simulink model "H175_V2_control"  (R2025b)
(part 2 of 12)

  ct_R_index3 : nesl_utility/Simulink-PS Converter  PhysicalDomain=network_engine_domain  SubClassName=ps_input  LeftPortType=input  RightPortType=output  PseudoPeriodic=off  Frequencies=[]  NoiseDistribution=none  NoiseParameters=[]  Unit=N*m  AffineConversion=off  FilteringAndDerivatives=provide  SimscapeFilterOrder=1  InputFilterTimeConstant=0.001  UdotUserProvided=0
  ct_R_little1 : nesl_utility/Simulink-PS Converter  PhysicalDomain=network_engine_domain  SubClassName=ps_input  LeftPortType=input  RightPortType=output  PseudoPeriodic=off  Frequencies=[]  NoiseDistribution=none  NoiseParameters=[]  Unit=N*m  AffineConversion=off  FilteringAndDerivatives=provide  SimscapeFilterOrder=1  InputFilterTimeConstant=0.001  UdotUserProvided=0
  ct_R_little2 : nesl_utility/Simulink-PS Converter  PhysicalDomain=network_engine_domain  SubClassName=ps_input  LeftPortType=input  RightPortType=output  PseudoPeriodic=off  Frequencies=[]  NoiseDistribution=none  NoiseParameters=[]  Unit=N*m  AffineConversion=off  FilteringAndDerivatives=provide  SimscapeFilterOrder=1  InputFilterTimeConstant=0.001  UdotUserProvided=0
  ct_R_little3 : nesl_utility/Simulink-PS Converter  PhysicalDomain=network_engine_domain  SubClassName=ps_input  LeftPortType=input  RightPortType=output  PseudoPeriodic=off  Frequencies=[]  NoiseDistribution=none  NoiseParameters=[]  Unit=N*m  AffineConversion=off  FilteringAndDerivatives=provide  SimscapeFilterOrder=1  InputFilterTimeConstant=0.001  UdotUserProvided=0
  ct_R_middle1 : nesl_utility/Simulink-PS Converter  PhysicalDomain=network_engine_domain  SubClassName=ps_input  LeftPortType=input  RightPortType=output  PseudoPeriodic=off  Frequencies=[]  NoiseDistribution=none  NoiseParameters=[]  Unit=N*m  AffineConversion=off  FilteringAndDerivatives=provide  SimscapeFilterOrder=1  InputFilterTimeConstant=0.001  UdotUserProvided=0
  ct_R_middle2 : nesl_utility/Simulink-PS Converter  PhysicalDomain=network_engine_domain  SubClassName=ps_input  LeftPortType=input  RightPortType=output  PseudoPeriodic=off  Frequencies=[]  NoiseDistribution=none  NoiseParameters=[]  Unit=N*m  AffineConversion=off  FilteringAndDerivatives=provide  SimscapeFilterOrder=1  InputFilterTimeConstant=0.001  UdotUserProvided=0
  ct_R_middle3 : nesl_utility/Simulink-PS Converter  PhysicalDomain=network_engine_domain  SubClassName=ps_input  LeftPortType=input  RightPortType=output  PseudoPeriodic=off  Frequencies=[]  NoiseDistribution=none  NoiseParameters=[]  Unit=N*m  AffineConversion=off  FilteringAndDerivatives=provide  SimscapeFilterOrder=1  InputFilterTimeConstant=0.001  UdotUserProvided=0
  ct_R_ring1 : nesl_utility/Simulink-PS Converter  PhysicalDomain=network_engine_domain  SubClassName=ps_input  LeftPortType=input  RightPortType=output  PseudoPeriodic=off  Frequencies=[]  NoiseDistribution=none  NoiseParameters=[]  Unit=N*m  AffineConversion=off  FilteringAndDerivatives=provide  SimscapeFilterOrder=1  InputFilterTimeConstant=0.001  UdotUserProvided=0
  ct_R_ring2 : nesl_utility/Simulink-PS Converter  PhysicalDomain=network_engine_domain  SubClassName=ps_input  LeftPortType=input  RightPortType=output  PseudoPeriodic=off  Frequencies=[]  NoiseDistribution=none  NoiseParameters=[]  Unit=N*m  AffineConversion=off  FilteringAndDerivatives=provide  SimscapeFilterOrder=1  InputFilterTimeConstant=0.001  UdotUserProvided=0
  ct_R_ring3 : nesl_utility/Simulink-PS Converter  PhysicalDomain=network_engine_domain  SubClassName=ps_input  LeftPortType=input  RightPortType=output  PseudoPeriodic=off  Frequencies=[]  NoiseDistribution=none  NoiseParameters=[]  Unit=N*m  AffineConversion=off  FilteringAndDerivatives=provide  SimscapeFilterOrder=1  InputFilterTimeConstant=0.001  UdotUserProvided=0
  ct_R_scapula : nesl_utility/Simulink-PS Converter  PhysicalDomain=network_engine_domain  SubClassName=ps_input  LeftPortType=input  RightPortType=output  PseudoPeriodic=off  Frequencies=[]  NoiseDistribution=none  NoiseParameters=[]  Unit=N*m  AffineConversion=off  FilteringAndDerivatives=provide  SimscapeFilterOrder=1  InputFilterTimeConstant=0.001  UdotUserProvided=0
  ct_R_shin : nesl_utility/Simulink-PS Converter  PhysicalDomain=network_engine_domain  SubClassName=ps_input  LeftPortType=input  RightPortType=output  PseudoPeriodic=off  Frequencies=[]  NoiseDistribution=none  NoiseParameters=[]  Unit=N*m  AffineConversion=off  FilteringAndDerivatives=provide  SimscapeFilterOrder=1  InputFilterTimeConstant=0.001  UdotUserProvided=0
  ct_R_shoulder_roll : nesl_utility/Simulink-PS Converter  PhysicalDomain=network_engine_domain  SubClassName=ps_input  LeftPortType=input  RightPortType=output  PseudoPeriodic=off  Frequencies=[]  NoiseDistribution=none  NoiseParameters=[]  Unit=N*m  AffineConversion=off  FilteringAndDerivatives=provide  SimscapeFilterOrder=1  InputFilterTimeConstant=0.001  UdotUserProvided=0
  ct_R_shoulder_yaw : nesl_utility/Simulink-PS Converter  PhysicalDomain=network_engine_domain  SubClassName=ps_input  LeftPortType=input  RightPortType=output  PseudoPeriodic=off  Frequencies=[]  NoiseDistribution=none  NoiseParameters=[]  Unit=N*m  AffineConversion=off  FilteringAndDerivatives=provide  SimscapeFilterOrder=1  InputFilterTimeConstant=0.001  UdotUserProvided=0
  ct_R_thigh : nesl_utility/Simulink-PS Converter  PhysicalDomain=network_engine_domain  SubClassName=ps_input  LeftPortType=input  RightPortType=output  PseudoPeriodic=off  Frequencies=[]  NoiseDistribution=none  NoiseParameters=[]  Unit=N*m  AffineConversion=off  FilteringAndDerivatives=provide  SimscapeFilterOrder=1  InputFilterTimeConstant=0.001  UdotUserProvided=0
  ct_R_thumb1 : nesl_utility/Simulink-PS Converter  PhysicalDomain=network_engine_domain  SubClassName=ps_input  LeftPortType=input  RightPortType=output  PseudoPeriodic=off  Frequencies=[]  NoiseDistribution=none  NoiseParameters=[]  Unit=N*m  AffineConversion=off  FilteringAndDerivatives=provide  SimscapeFilterOrder=1  InputFilterTimeConstant=0.001  UdotUserProvided=0
  ct_R_thumb2 : nesl_utility/Simulink-PS Converter  PhysicalDomain=network_engine_domain  SubClassName=ps_input  LeftPortType=input  RightPortType=output  PseudoPeriodic=off  Frequencies=[]  NoiseDistribution=none  NoiseParameters=[]  Unit=N*m  AffineConversion=off  FilteringAndDerivatives=provide  SimscapeFilterOrder=1  InputFilterTimeConstant=0.001  UdotUserProvided=0
  ct_R_thumb3 : nesl_utility/Simulink-PS Converter  PhysicalDomain=network_engine_domain  SubClassName=ps_input  LeftPortType=input  RightPortType=output  PseudoPeriodic=off  Frequencies=[]  NoiseDistribution=none  NoiseParameters=[]  Unit=N*m  AffineConversion=off  FilteringAndDerivatives=provide  SimscapeFilterOrder=1  InputFilterTimeConstant=0.001  UdotUserProvided=0
  ct_R_toe : nesl_utility/Simulink-PS Converter  PhysicalDomain=network_engine_domain  SubClassName=ps_input  LeftPortType=input  RightPortType=output  PseudoPeriodic=off  Frequencies=[]  NoiseDistribution=none  NoiseParameters=[]  Unit=N*m  AffineConversion=off  FilteringAndDerivatives=provide  SimscapeFilterOrder=1  InputFilterTimeConstant=0.001  UdotUserProvided=0
  ct_R_upper_arm : nesl_utility/Simulink-PS Converter  PhysicalDomain=network_engine_domain  SubClassName=ps_input  LeftPortType=input  RightPortType=output  PseudoPeriodic=off  Frequencies=[]  NoiseDistribution=none  NoiseParameters=[]  Unit=N*m  AffineConversion=off  FilteringAndDerivatives=provide  SimscapeFilterOrder=1  InputFilterTimeConstant=0.001  UdotUserProvided=0
  ct_R_wrist_roll : nesl_utility/Simulink-PS Converter  PhysicalDomain=network_engine_domain  SubClassName=ps_input  LeftPortType=input  RightPortType=output  PseudoPeriodic=off  Frequencies=[]  NoiseDistribution=none  NoiseParameters=[]  Unit=N*m  AffineConversion=off  FilteringAndDerivatives=provide  SimscapeFilterOrder=1  InputFilterTimeConstant=0.001  UdotUserProvided=0
  ct_R_wrist_yaw : nesl_utility/Simulink-PS Converter  PhysicalDomain=network_engine_domain  SubClassName=ps_input  LeftPortType=input  RightPortType=output  PseudoPeriodic=off  Frequencies=[]  NoiseDistribution=none  NoiseParameters=[]  Unit=N*m  AffineConversion=off  FilteringAndDerivatives=provide  SimscapeFilterOrder=1  InputFilterTimeConstant=0.001  UdotUserProvided=0
  ct_neck_pitch : nesl_utility/Simulink-PS Converter  PhysicalDomain=network_engine_domain  SubClassName=ps_input  LeftPortType=input  RightPortType=output  PseudoPeriodic=off  Frequencies=[]  NoiseDistribution=none  NoiseParameters=[]  Unit=N*m  AffineConversion=off  FilteringAndDerivatives=provide  SimscapeFilterOrder=1  InputFilterTimeConstant=0.001  UdotUserProvided=0
  ct_neck_roll : nesl_utility/Simulink-PS Converter  PhysicalDomain=network_engine_domain  SubClassName=ps_input  LeftPortType=input  RightPortType=output  PseudoPeriodic=off  Frequencies=[]  NoiseDistribution=none  NoiseParameters=[]  Unit=N*m  AffineConversion=off  FilteringAndDerivatives=provide  SimscapeFilterOrder=1  InputFilterTimeConstant=0.001  UdotUserProvided=0
  ct_neck_yaw : nesl_utility/Simulink-PS Converter  PhysicalDomain=network_engine_domain  SubClassName=ps_input  LeftPortType=input  RightPortType=output  PseudoPeriodic=off  Frequencies=[]  NoiseDistribution=none  NoiseParameters=[]  Unit=N*m  AffineConversion=off  FilteringAndDerivatives=provide  SimscapeFilterOrder=1  InputFilterTimeConstant=0.001  UdotUserProvided=0
  ct_waist_pitch : nesl_utility/Simulink-PS Converter  PhysicalDomain=network_engine_domain  SubClassName=ps_input  LeftPortType=input  RightPortType=output  PseudoPeriodic=off  Frequencies=[]  NoiseDistribution=none  NoiseParameters=[]  Unit=N*m  AffineConversion=off  FilteringAndDerivatives=provide  SimscapeFilterOrder=1  InputFilterTimeConstant=0.001  UdotUserProvided=0
  ct_waist_roll : nesl_utility/Simulink-PS Converter  PhysicalDomain=network_engine_domain  SubClassName=ps_input  LeftPortType=input  RightPortType=output  PseudoPeriodic=off  Frequencies=[]  NoiseDistribution=none  NoiseParameters=[]  Unit=N*m  AffineConversion=off  FilteringAndDerivatives=provide  SimscapeFilterOrder=1  InputFilterTimeConstant=0.001  UdotUserProvided=0
  ct_waist_yaw : nesl_utility/Simulink-PS Converter  PhysicalDomain=network_engine_domain  SubClassName=ps_input  LeftPortType=input  RightPortType=output  PseudoPeriodic=off  Frequencies=[]  NoiseDistribution=none  NoiseParameters=[]  Unit=N*m  AffineConversion=off  FilteringAndDerivatives=provide  SimscapeFilterOrder=1  InputFilterTimeConstant=0.001  UdotUserProvided=0
  cw_L_ankle_pitch : nesl_utility/PS-Simulink Converter  PhysicalDomain=network_engine_domain  SubClassName=ps_output  LeftPortType=input  RightPortType=output  PseudoPeriodic=off  Frequencies=[]  VectorFormat=inherit  Unit=rad/s  AffineConversion=off
  cw_L_arm_twist : nesl_utility/PS-Simulink Converter  PhysicalDomain=network_engine_domain  SubClassName=ps_output  LeftPortType=input  RightPortType=output  PseudoPeriodic=off  Frequencies=[]  VectorFormat=inherit  Unit=rad/s  AffineConversion=off
  cw_L_foot : nesl_utility/PS-Simulink Converter  PhysicalDomain=network_engine_domain  SubClassName=ps_output  LeftPortType=input  RightPortType=output  PseudoPeriodic=off  Frequencies=[]  VectorFormat=inherit  Unit=rad/s  AffineConversion=off
  cw_L_forearm : nesl_utility/PS-Simulink Converter  PhysicalDomain=network_engine_domain  SubClassName=ps_output  LeftPortType=input  RightPortType=output  PseudoPeriodic=off  Frequencies=[]  VectorFormat=inherit  Unit=rad/s  AffineConversion=off
  cw_L_forearm_twist : nesl_utility/PS-Simulink Converter  PhysicalDomain=network_engine_domain  SubClassName=ps_output  LeftPortType=input  RightPortType=output  PseudoPeriodic=off  Frequencies=[]  VectorFormat=inherit  Unit=rad/s  AffineConversion=off
  cw_L_hand : nesl_utility/PS-Simulink Converter  PhysicalDomain=network_engine_domain  SubClassName=ps_output  LeftPortType=input  RightPortType=output  PseudoPeriodic=off  Frequencies=[]  VectorFormat=inherit  Unit=rad/s  AffineConversion=off
  cw_L_hip_aux : nesl_utility/PS-Simulink Converter  PhysicalDomain=network_engine_domain  SubClassName=ps_output  LeftPortType=input  RightPortType=output  PseudoPeriodic=off  Frequencies=[]  VectorFormat=inherit  Unit=rad/s  AffineConversion=off
  cw_L_hip_roll : nesl_utility/PS-Simulink Converter  PhysicalDomain=network_engine_domain  SubClassName=ps_output  LeftPortType=input  RightPortType=output  PseudoPeriodic=off  Frequencies=[]  VectorFormat=inherit  Unit=rad/s  AffineConversion=off
  cw_L_hip_yaw : nesl_utility/PS-Simulink Converter  PhysicalDomain=network_engine_domain  SubClassName=ps_output  LeftPortType=input  RightPortType=output  PseudoPeriodic=off  Frequencies=[]  VectorFormat=inherit  Unit=rad/s  AffineConversion=off
  cw_L_index1 : nesl_utility/PS-Simulink Converter  PhysicalDomain=network_engine_domain  SubClassName=ps_output  LeftPortType=input  RightPortType=output  PseudoPeriodic=off  Frequencies=[]  VectorFormat=inherit  Unit=rad/s  AffineConversion=off
  cw_L_index2 : nesl_utility/PS-Simulink Converter  PhysicalDomain=network_engine_domain  SubClassName=ps_output  LeftPortType=input  RightPortType=output  PseudoPeriodic=off  Frequencies=[]  VectorFormat=inherit  Unit=rad/s  AffineConversion=off
  cw_L_index3 : nesl_utility/PS-Simulink Converter  PhysicalDomain=network_engine_domain  SubClassName=ps_output  LeftPortType=input  RightPortType=output  PseudoPeriodic=off  Frequencies=[]  VectorFormat=inherit  Unit=rad/s  AffineConversion=off
  cw_L_little1 : nesl_utility/PS-Simulink Converter  PhysicalDomain=network_engine_domain  SubClassName=ps_output  LeftPortType=input  RightPortType=output  PseudoPeriodic=off  Frequencies=[]  VectorFormat=inherit  Unit=rad/s  AffineConversion=off
  cw_L_little2 : nesl_utility/PS-Simulink Converter  PhysicalDomain=network_engine_domain  SubClassName=ps_output  LeftPortType=input  RightPortType=output  PseudoPeriodic=off  Frequencies=[]  VectorFormat=inherit  Unit=rad/s  AffineConversion=off
  cw_L_little3 : nesl_utility/PS-Simulink Converter  PhysicalDomain=network_engine_domain  SubClassName=ps_output  LeftPortType=input  RightPortType=output  PseudoPeriodic=off  Frequencies=[]  VectorFormat=inherit  Unit=rad/s  AffineConversion=off
  cw_L_middle1 : nesl_utility/PS-Simulink Converter  PhysicalDomain=network_engine_domain  SubClassName=ps_output  LeftPortType=input  RightPortType=output  PseudoPeriodic=off  Frequencies=[]  VectorFormat=inherit  Unit=rad/s  AffineConversion=off
  cw_L_middle2 : nesl_utility/PS-Simulink Converter  PhysicalDomain=network_engine_domain  SubClassName=ps_output  LeftPortType=input  RightPortType=output  PseudoPeriodic=off  Frequencies=[]  VectorFormat=inherit  Unit=rad/s  AffineConversion=off
  cw_L_middle3 : nesl_utility/PS-Simulink Converter  PhysicalDomain=network_engine_domain  SubClassName=ps_output  LeftPortType=input  RightPortType=output  PseudoPeriodic=off  Frequencies=[]  VectorFormat=inherit  Unit=rad/s  AffineConversion=off
  cw_L_ring1 : nesl_utility/PS-Simulink Converter  PhysicalDomain=network_engine_domain  SubClassName=ps_output  LeftPortType=input  RightPortType=output  PseudoPeriodic=off  Frequencies=[]  VectorFormat=inherit  Unit=rad/s  AffineConversion=off
  cw_L_ring2 : nesl_utility/PS-Simulink Converter  PhysicalDomain=network_engine_domain  SubClassName=ps_output  LeftPortType=input  RightPortType=output  PseudoPeriodic=off  Frequencies=[]  VectorFormat=inherit  Unit=rad/s  AffineConversion=off
  cw_L_ring3 : nesl_utility/PS-Simulink Converter  PhysicalDomain=network_engine_domain  SubClassName=ps_output  LeftPortType=input  RightPortType=output  PseudoPeriodic=off  Frequencies=[]  VectorFormat=inherit  Unit=rad/s  AffineConversion=off
  cw_L_scapula : nesl_utility/PS-Simulink Converter  PhysicalDomain=network_engine_domain  SubClassName=ps_output  LeftPortType=input  RightPortType=output  PseudoPeriodic=off  Frequencies=[]  VectorFormat=inherit  Unit=rad/s  AffineConversion=off
  cw_L_shin : nesl_utility/PS-Simulink Converter  PhysicalDomain=network_engine_domain  SubClassName=ps_output  LeftPortType=input  RightPortType=output  PseudoPeriodic=off  Frequencies=[]  VectorFormat=inherit  Unit=rad/s  AffineConversion=off
  cw_L_shoulder_roll : nesl_utility/PS-Simulink Converter  PhysicalDomain=network_engine_domain  SubClassName=ps_output  LeftPortType=input  RightPortType=output  PseudoPeriodic=off  Frequencies=[]  VectorFormat=inherit  Unit=rad/s  AffineConversion=off
  cw_L_shoulder_yaw : nesl_utility/PS-Simulink Converter  PhysicalDomain=network_engine_domain  SubClassName=ps_output  LeftPortType=input  RightPortType=output  PseudoPeriodic=off  Frequencies=[]  VectorFormat=inherit  Unit=rad/s  AffineConversion=off
  cw_L_thigh : nesl_utility/PS-Simulink Converter  PhysicalDomain=network_engine_domain  SubClassName=ps_output  LeftPortType=input  RightPortType=output  PseudoPeriodic=off  Frequencies=[]  VectorFormat=inherit  Unit=rad/s  AffineConversion=off
  cw_L_thumb1 : nesl_utility/PS-Simulink Converter  PhysicalDomain=network_engine_domain  SubClassName=ps_output  LeftPortType=input  RightPortType=output  PseudoPeriodic=off  Frequencies=[]  VectorFormat=inherit  Unit=rad/s  AffineConversion=off
  cw_L_thumb2 : nesl_utility/PS-Simulink Converter  PhysicalDomain=network_engine_domain  SubClassName=ps_output  LeftPortType=input  RightPortType=output  PseudoPeriodic=off  Frequencies=[]  VectorFormat=inherit  Unit=rad/s  AffineConversion=off
  cw_L_thumb3 : nesl_utility/PS-Simulink Converter  PhysicalDomain=network_engine_domain  SubClassName=ps_output  LeftPortType=input  RightPortType=output  PseudoPeriodic=off  Frequencies=[]  VectorFormat=inherit  Unit=rad/s  AffineConversion=off
  cw_L_toe : nesl_utility/PS-Simulink Converter  PhysicalDomain=network_engine_domain  SubClassName=ps_output  LeftPortType=input  RightPortType=output  PseudoPeriodic=off  Frequencies=[]  VectorFormat=inherit  Unit=rad/s  AffineConversion=off
  cw_L_upper_arm : nesl_utility/PS-Simulink Converter  PhysicalDomain=network_engine_domain  SubClassName=ps_output  LeftPortType=input  RightPortType=output  PseudoPeriodic=off  Frequencies=[]  VectorFormat=inherit  Unit=rad/s  AffineConversion=off
  cw_L_wrist_roll : nesl_utility/PS-Simulink Converter  PhysicalDomain=network_engine_domain  SubClassName=ps_output  LeftPortType=input  RightPortType=output  PseudoPeriodic=off  Frequencies=[]  VectorFormat=inherit  Unit=rad/s  AffineConversion=off
  cw_L_wrist_yaw : nesl_utility/PS-Simulink Converter  PhysicalDomain=network_engine_domain  SubClassName=ps_output  LeftPortType=input  RightPortType=output  PseudoPeriodic=off  Frequencies=[]  VectorFormat=inherit  Unit=rad/s  AffineConversion=off
  cw_R_ankle_pitch : nesl_utility/PS-Simulink Converter  PhysicalDomain=network_engine_domain  SubClassName=ps_output  LeftPortType=input  RightPortType=output  PseudoPeriodic=off  Frequencies=[]  VectorFormat=inherit  Unit=rad/s  AffineConversion=off
  cw_R_arm_twist : nesl_utility/PS-Simulink Converter  PhysicalDomain=network_engine_domain  SubClassName=ps_output  LeftPortType=input  RightPortType=output  PseudoPeriodic=off  Frequencies=[]  VectorFormat=inherit  Unit=rad/s  AffineConversion=off
  cw_R_foot : nesl_utility/PS-Simulink Converter  PhysicalDomain=network_engine_domain  SubClassName=ps_output  LeftPortType=input  RightPortType=output  PseudoPeriodic=off  Frequencies=[]  VectorFormat=inherit  Unit=rad/s  AffineConversion=off
  cw_R_forearm : nesl_utility/PS-Simulink Converter  PhysicalDomain=network_engine_domain  SubClassName=ps_output  LeftPortType=input  RightPortType=output  PseudoPeriodic=off  Frequencies=[]  VectorFormat=inherit  Unit=rad/s  AffineConversion=off
  cw_R_forearm_twist : nesl_utility/PS-Simulink Converter  PhysicalDomain=network_engine_domain  SubClassName=ps_output  LeftPortType=input  RightPortType=output  PseudoPeriodic=off  Frequencies=[]  VectorFormat=inherit  Unit=rad/s  AffineConversion=off
  cw_R_hand : nesl_utility/PS-Simulink Converter  PhysicalDomain=network_engine_domain  SubClassName=ps_output  LeftPortType=input  RightPortType=output  PseudoPeriodic=off  Frequencies=[]  VectorFormat=inherit  Unit=rad/s  AffineConversion=off
  cw_R_hip_aux : nesl_utility/PS-Simulink Converter  PhysicalDomain=network_engine_domain  SubClassName=ps_output  LeftPortType=input  RightPortType=output  PseudoPeriodic=off  Frequencies=[]  VectorFormat=inherit  Unit=rad/s  AffineConversion=off
  cw_R_hip_roll : nesl_utility/PS-Simulink Converter  PhysicalDomain=network_engine_domain  SubClassName=ps_output  LeftPortType=input  RightPortType=output  PseudoPeriodic=off  Frequencies=[]  VectorFormat=inherit  Unit=rad/s  AffineConversion=off
  cw_R_hip_yaw : nesl_utility/PS-Simulink Converter  PhysicalDomain=network_engine_domain  SubClassName=ps_output  LeftPortType=input  RightPortType=output  PseudoPeriodic=off  Frequencies=[]  VectorFormat=inherit  Unit=rad/s  AffineConversion=off
  cw_R_index1 : nesl_utility/PS-Simulink Converter  PhysicalDomain=network_engine_domain  SubClassName=ps_output  LeftPortType=input  RightPortType=output  PseudoPeriodic=off  Frequencies=[]  VectorFormat=inherit  Unit=rad/s  AffineConversion=off
  cw_R_index2 : nesl_utility/PS-Simulink Converter  PhysicalDomain=network_engine_domain  SubClassName=ps_output  LeftPortType=input  RightPortType=output  PseudoPeriodic=off  Frequencies=[]  VectorFormat=inherit  Unit=rad/s  AffineConversion=off
  cw_R_index3 : nesl_utility/PS-Simulink Converter  PhysicalDomain=network_engine_domain  SubClassName=ps_output  LeftPortType=input  RightPortType=output  PseudoPeriodic=off  Frequencies=[]  VectorFormat=inherit  Unit=rad/s  AffineConversion=off
  cw_R_little1 : nesl_utility/PS-Simulink Converter  PhysicalDomain=network_engine_domain  SubClassName=ps_output  LeftPortType=input  RightPortType=output  PseudoPeriodic=off  Frequencies=[]  VectorFormat=inherit  Unit=rad/s  AffineConversion=off
  cw_R_little2 : nesl_utility/PS-Simulink Converter  PhysicalDomain=network_engine_domain  SubClassName=ps_output  LeftPortType=input  RightPortType=output  PseudoPeriodic=off  Frequencies=[]  VectorFormat=inherit  Unit=rad/s  AffineConversion=off
  cw_R_little3 : nesl_utility/PS-Simulink Converter  PhysicalDomain=network_engine_domain  SubClassName=ps_output  LeftPortType=input  RightPortType=output  PseudoPeriodic=off  Frequencies=[]  VectorFormat=inherit  Unit=rad/s  AffineConversion=off
  cw_R_middle1 : nesl_utility/PS-Simulink Converter  PhysicalDomain=network_engine_domain  SubClassName=ps_output  LeftPortType=input  RightPortType=output  PseudoPeriodic=off  Frequencies=[]  VectorFormat=inherit  Unit=rad/s  AffineConversion=off
  cw_R_middle2 : nesl_utility/PS-Simulink Converter  PhysicalDomain=network_engine_domain  SubClassName=ps_output  LeftPortType=input  RightPortType=output  PseudoPeriodic=off  Frequencies=[]  VectorFormat=inherit  Unit=rad/s  AffineConversion=off
  cw_R_middle3 : nesl_utility/PS-Simulink Converter  PhysicalDomain=network_engine_domain  SubClassName=ps_output  LeftPortType=input  RightPortType=output  PseudoPeriodic=off  Frequencies=[]  VectorFormat=inherit  Unit=rad/s  AffineConversion=off
  cw_R_ring1 : nesl_utility/PS-Simulink Converter  PhysicalDomain=network_engine_domain  SubClassName=ps_output  LeftPortType=input  RightPortType=output  PseudoPeriodic=off  Frequencies=[]  VectorFormat=inherit  Unit=rad/s  AffineConversion=off
  cw_R_ring2 : nesl_utility/PS-Simulink Converter  PhysicalDomain=network_engine_domain  SubClassName=ps_output  LeftPortType=input  RightPortType=output  PseudoPeriodic=off  Frequencies=[]  VectorFormat=inherit  Unit=rad/s  AffineConversion=off
  cw_R_ring3 : nesl_utility/PS-Simulink Converter  PhysicalDomain=network_engine_domain  SubClassName=ps_output  LeftPortType=input  RightPortType=output  PseudoPeriodic=off  Frequencies=[]  VectorFormat=inherit  Unit=rad/s  AffineConversion=off
  cw_R_scapula : nesl_utility/PS-Simulink Converter  PhysicalDomain=network_engine_domain  SubClassName=ps_output  LeftPortType=input  RightPortType=output  PseudoPeriodic=off  Frequencies=[]  VectorFormat=inherit  Unit=rad/s  AffineConversion=off
  cw_R_shin : nesl_utility/PS-Simulink Converter  PhysicalDomain=network_engine_domain  SubClassName=ps_output  LeftPortType=input  RightPortType=output  PseudoPeriodic=off  Frequencies=[]  VectorFormat=inherit  Unit=rad/s  AffineConversion=off
  cw_R_shoulder_roll : nesl_utility/PS-Simulink Converter  PhysicalDomain=network_engine_domain  SubClassName=ps_output  LeftPortType=input  RightPortType=output  PseudoPeriodic=off  Frequencies=[]  VectorFormat=inherit  Unit=rad/s  AffineConversion=off
  cw_R_shoulder_yaw : nesl_utility/PS-Simulink Converter  PhysicalDomain=network_engine_domain  SubClassName=ps_output  LeftPortType=input  RightPortType=output  PseudoPeriodic=off  Frequencies=[]  VectorFormat=inherit  Unit=rad/s  AffineConversion=off
  cw_R_thigh : nesl_utility/PS-Simulink Converter  PhysicalDomain=network_engine_domain  SubClassName=ps_output  LeftPortType=input  RightPortType=output  PseudoPeriodic=off  Frequencies=[]  VectorFormat=inherit  Unit=rad/s  AffineConversion=off
  cw_R_thumb1 : nesl_utility/PS-Simulink Converter  PhysicalDomain=network_engine_domain  SubClassName=ps_output  LeftPortType=input  RightPortType=output  PseudoPeriodic=off  Frequencies=[]  VectorFormat=inherit  Unit=rad/s  AffineConversion=off
  cw_R_thumb2 : nesl_utility/PS-Simulink Converter  PhysicalDomain=network_engine_domain  SubClassName=ps_output  LeftPortType=input  RightPortType=output  PseudoPeriodic=off  Frequencies=[]  VectorFormat=inherit  Unit=rad/s  AffineConversion=off
  cw_R_thumb3 : nesl_utility/PS-Simulink Converter  PhysicalDomain=network_engine_domain  SubClassName=ps_output  LeftPortType=input  RightPortType=output  PseudoPeriodic=off  Frequencies=[]  VectorFormat=inherit  Unit=rad/s  AffineConversion=off
  cw_R_toe : nesl_utility/PS-Simulink Converter  PhysicalDomain=network_engine_domain  SubClassName=ps_output  LeftPortType=input  RightPortType=output  PseudoPeriodic=off  Frequencies=[]  VectorFormat=inherit  Unit=rad/s  AffineConversion=off
  cw_R_upper_arm : nesl_utility/PS-Simulink Converter  PhysicalDomain=network_engine_domain  SubClassName=ps_output  LeftPortType=input  RightPortType=output  PseudoPeriodic=off  Frequencies=[]  VectorFormat=inherit  Unit=rad/s  AffineConversion=off
  cw_R_wrist_roll : nesl_utility/PS-Simulink Converter  PhysicalDomain=network_engine_domain  SubClassName=ps_output  LeftPortType=input  RightPortType=output  PseudoPeriodic=off  Frequencies=[]  VectorFormat=inherit  Unit=rad/s  AffineConversion=off
  cw_R_wrist_yaw : nesl_utility/PS-Simulink Converter  PhysicalDomain=network_engine_domain  SubClassName=ps_output  LeftPortType=input  RightPortType=output  PseudoPeriodic=off  Frequencies=[]  VectorFormat=inherit  Unit=rad/s  AffineConversion=off
  cw_neck_pitch : nesl_utility/PS-Simulink Converter  PhysicalDomain=network_engine_domain  SubClassName=ps_output  LeftPortType=input  RightPortType=output  PseudoPeriodic=off  Frequencies=[]  VectorFormat=inherit  Unit=rad/s  AffineConversion=off
  cw_neck_roll : nesl_utility/PS-Simulink Converter  PhysicalDomain=network_engine_domain  SubClassName=ps_output  LeftPortType=input  RightPortType=output  PseudoPeriodic=off  Frequencies=[]  VectorFormat=inherit  Unit=rad/s  AffineConversion=off
  cw_neck_yaw : nesl_utility/PS-Simulink Converter  PhysicalDomain=network_engine_domain  SubClassName=ps_output  LeftPortType=input  RightPortType=output  PseudoPeriodic=off  Frequencies=[]  VectorFormat=inherit  Unit=rad/s  AffineConversion=off
  cw_waist_pitch : nesl_utility/PS-Simulink Converter  PhysicalDomain=network_engine_domain  SubClassName=ps_output  LeftPortType=input  RightPortType=output  PseudoPeriodic=off  Frequencies=[]  VectorFormat=inherit  Unit=rad/s  AffineConversion=off
  cw_waist_roll : nesl_utility/PS-Simulink Converter  PhysicalDomain=network_engine_domain  SubClassName=ps_output  LeftPortType=input  RightPortType=output  PseudoPeriodic=off  Frequencies=[]  VectorFormat=inherit  Unit=rad/s  AffineConversion=off
  cw_waist_yaw : nesl_utility/PS-Simulink Converter  PhysicalDomain=network_engine_domain  SubClassName=ps_output  LeftPortType=input  RightPortType=output  PseudoPeriodic=off  Frequencies=[]  VectorFormat=inherit  Unit=rad/s  AffineConversion=off
  head : Subsystem
  neck_pitch : sm_lib/Joints/Revolute Joint  JointMode=Normal  CompositeWrenchDir=FollowerOnBase  CompositeWrenchFrame=BaseFrame  SenseConstraintForce=off  SenseConstraintTorque=off  SenseTotalForce=off  SenseTotalTorque=off  PositionTargetSpecify=off  PositionTargetPriority=High  PositionTargetValue=0  PositionTargetValueUnits=deg  VelocityTargetSpecify=off  VelocityTargetPriority=High  VelocityTargetValue=0  VelocityTargetValueUnits=deg/s  EquilibriumPosition=0  EquilibriumPositionUnits=deg  SpringStiffness=0  SpringStiffnessUnits=N*m/deg  DampingCoefficient=0  DampingCoefficientUnits=kg*m^2/(rad*s)  LowerLimitSpecify=on  LowerLimitBound=-0.6108652381980153  LowerLimitBoundUnits=rad  LowerLimitStiffness=1e4  LowerLimitStiffnessUnits=N*m/deg  LowerLimitDamping=10  LowerLimitDampingUnits=N*m/(deg/s)  LowerLimitTransitionRegionWidth=0.1  LowerLimitTransitionRegionWidthUnits=deg  UpperLimitSpecify=on  UpperLimitBound=0.6108652381980153  UpperLimitBoundUnits=rad  UpperLimitStiffness=1e4  UpperLimitStiffnessUnits=N*m/deg  UpperLimitDamping=10  UpperLimitDampingUnits=N*m/(deg/s)  UpperLimitTransitionRegionWidth=0.1  UpperLimitTransitionRegionWidthUnits=deg  TorqueActuationMode=InputTorque  MotionActuationMode=ComputedMotion  SensePosition=on  SenseVelocity=on  SenseAcceleration=off  SenseTorqueForce=off  SenseLowerLimitTorqueForce=off  SenseUpperLimitTorqueForce=off
  neck_roll : sm_lib/Joints/Revolute Joint  JointMode=Normal  CompositeWrenchDir=FollowerOnBase  CompositeWrenchFrame=BaseFrame  SenseConstraintForce=off  SenseConstraintTorque=off  SenseTotalForce=off  SenseTotalTorque=off  PositionTargetSpecify=off  PositionTargetPriority=High  PositionTargetValue=0  PositionTargetValueUnits=deg  VelocityTargetSpecify=off  VelocityTargetPriority=High  VelocityTargetValue=0  VelocityTargetValueUnits=deg/s  EquilibriumPosition=0  EquilibriumPositionUnits=deg  SpringStiffness=0  SpringStiffnessUnits=N*m/deg  DampingCoefficient=0  DampingCoefficientUnits=kg*m^2/(rad*s)  LowerLimitSpecify=on  LowerLimitBound=-0.3490658503988659  LowerLimitBoundUnits=rad  LowerLimitStiffness=1e4  LowerLimitStiffnessUnits=N*m/deg  LowerLimitDamping=10  LowerLimitDampingUnits=N*m/(deg/s)  LowerLimitTransitionRegionWidth=0.1  LowerLimitTransitionRegionWidthUnits=deg  UpperLimitSpecify=on  UpperLimitBound=0.3490658503988659  UpperLimitBoundUnits=rad  UpperLimitStiffness=1e4  UpperLimitStiffnessUnits=N*m/deg  UpperLimitDamping=10  UpperLimitDampingUnits=N*m/(deg/s)  UpperLimitTransitionRegionWidth=0.1  UpperLimitTransitionRegionWidthUnits=deg  TorqueActuationMode=InputTorque  MotionActuationMode=ComputedMotion  SensePosition=on  SenseVelocity=on  SenseAcceleration=off  SenseTorqueForce=off  SenseLowerLimitTorqueForce=off  SenseUpperLimitTorqueForce=off
  neck_roll1 : Subsystem
  neck_yaw : sm_lib/Joints/Revolute Joint  JointMode=Normal  CompositeWrenchDir=FollowerOnBase  CompositeWrenchFrame=BaseFrame  SenseConstraintForce=off  SenseConstraintTorque=off  SenseTotalForce=off  SenseTotalTorque=off  PositionTargetSpecify=off  PositionTargetPriority=High  PositionTargetValue=0  PositionTargetValueUnits=deg  VelocityTargetSpecify=off  VelocityTargetPriority=High  VelocityTargetValue=0  VelocityTargetValueUnits=deg/s  EquilibriumPosition=0  EquilibriumPositionUnits=deg  SpringStiffness=0  SpringStiffnessUnits=N*m/deg  DampingCoefficient=0  DampingCoefficientUnits=kg*m^2/(rad*s)  LowerLimitSpecify=on  LowerLimitBound=-1.48352986419518  LowerLimitBoundUnits=rad  LowerLimitStiffness=1e4  LowerLimitStiffnessUnits=N*m/deg  LowerLimitDamping=10  LowerLimitDampingUnits=N*m/(deg/s)  LowerLimitTransitionRegionWidth=0.1  LowerLimitTransitionRegionWidthUnits=deg  UpperLimitSpecify=on  UpperLimitBound=1.48352986419518  UpperLimitBoundUnits=rad  UpperLimitStiffness=1e4  UpperLimitStiffnessUnits=N*m/deg  UpperLimitDamping=10  UpperLimitDampingUnits=N*m/(deg/s)  UpperLimitTransitionRegionWidth=0.1  UpperLimitTransitionRegionWidthUnits=deg  TorqueActuationMode=InputTorque  MotionActuationMode=ComputedMotion  SensePosition=on  SenseVelocity=on  SenseAcceleration=off  SenseTorqueForce=off  SenseLowerLimitTorqueForce=off  SenseUpperLimitTorqueForce=off
  neck_yaw1 : Subsystem
  pelvis : Subsystem
  qref : FromWorkspace  VariableName=qref  OutputAfterFinalValue=Holding final value
  qref_demux : Demux  Outputs=72
  torso : Subsystem
  waist_pitch : sm_lib/Joints/Revolute Joint  JointMode=Normal  CompositeWrenchDir=FollowerOnBase  CompositeWrenchFrame=BaseFrame  SenseConstraintForce=off  SenseConstraintTorque=off  SenseTotalForce=off  SenseTotalTorque=off  PositionTargetSpecify=off  PositionTargetPriority=High  PositionTargetValue=0  PositionTargetValueUnits=deg  VelocityTargetSpecify=off  VelocityTargetPriority=High  VelocityTargetValue=0  VelocityTargetValueUnits=deg/s  EquilibriumPosition=0  EquilibriumPositionUnits=deg  SpringStiffness=0  SpringStiffnessUnits=N*m/deg  DampingCoefficient=0  DampingCoefficientUnits=kg*m^2/(rad*s)  LowerLimitSpecify=on  LowerLimitBound=-0.5235987755982988  LowerLimitBoundUnits=rad  LowerLimitStiffness=1e4  LowerLimitStiffnessUnits=N*m/deg  LowerLimitDamping=10  LowerLimitDampingUnits=N*m/(deg/s)  LowerLimitTransitionRegionWidth=0.1  LowerLimitTransitionRegionWidthUnits=deg  UpperLimitSpecify=on  UpperLimitBound=0.7853981633974483  UpperLimitBoundUnits=rad  UpperLimitStiffness=1e4  UpperLimitStiffnessUnits=N*m/deg  UpperLimitDamping=10  UpperLimitDampingUnits=N*m/(deg/s)  UpperLimitTransitionRegionWidth=0.1  UpperLimitTransitionRegionWidthUnits=deg  TorqueActuationMode=InputTorque  MotionActuationMode=ComputedMotion  SensePosition=on  SenseVelocity=on  SenseAcceleration=off  SenseTorqueForce=off  SenseLowerLimitTorqueForce=off  SenseUpperLimitTorqueForce=off
  waist_roll : sm_lib/Joints/Revolute Joint  JointMode=Normal  CompositeWrenchDir=FollowerOnBase  CompositeWrenchFrame=BaseFrame  SenseConstraintForce=off  SenseConstraintTorque=off  SenseTotalForce=off  SenseTotalTorque=off  PositionTargetSpecify=off  PositionTargetPriority=High  PositionTargetValue=0  PositionTargetValueUnits=deg  VelocityTargetSpecify=off  VelocityTargetPriority=High  VelocityTargetValue=0  VelocityTargetValueUnits=deg/s  EquilibriumPosition=0  EquilibriumPositionUnits=deg  SpringStiffness=0  SpringStiffnessUnits=N*m/deg  DampingCoefficient=0  DampingCoefficientUnits=kg*m^2/(rad*s)  LowerLimitSpecify=on  LowerLimitBound=-0.3490658503988659  LowerLimitBoundUnits=rad  LowerLimitStiffness=1e4  LowerLimitStiffnessUnits=N*m/deg  LowerLimitDamping=10  LowerLimitDampingUnits=N*m/(deg/s)  LowerLimitTransitionRegionWidth=0.1  LowerLimitTransitionRegionWidthUnits=deg  UpperLimitSpecify=on  UpperLimitBound=0.3490658503988659  UpperLimitBoundUnits=rad  UpperLimitStiffness=1e4  UpperLimitStiffnessUnits=N*m/deg  UpperLimitDamping=10  UpperLimitDampingUnits=N*m/(deg/s)  UpperLimitTransitionRegionWidth=0.1  UpperLimitTransitionRegionWidthUnits=deg  TorqueActuationMode=InputTorque  MotionActuationMode=ComputedMotion  SensePosition=on  SenseVelocity=on  SenseAcceleration=off  SenseTorqueForce=off  SenseLowerLimitTorqueForce=off  SenseUpperLimitTorqueForce=off
  waist_roll1 : Subsystem
  waist_yaw : sm_lib/Joints/Revolute Joint  JointMode=Normal  CompositeWrenchDir=FollowerOnBase  CompositeWrenchFrame=BaseFrame  SenseConstraintForce=off  SenseConstraintTorque=off  SenseTotalForce=off  SenseTotalTorque=off  PositionTargetSpecify=off  PositionTargetPriority=High  PositionTargetValue=0  PositionTargetValueUnits=deg  VelocityTargetSpecify=off  VelocityTargetPriority=High  VelocityTargetValue=0  VelocityTargetValueUnits=deg/s  EquilibriumPosition=0  EquilibriumPositionUnits=deg  SpringStiffness=0  SpringStiffnessUnits=N*m/deg  DampingCoefficient=0  DampingCoefficientUnits=kg*m^2/(rad*s)  LowerLimitSpecify=on  LowerLimitBound=-1.047197551196598  LowerLimitBoundUnits=rad  LowerLimitStiffness=1e4  LowerLimitStiffnessUnits=N*m/deg  LowerLimitDamping=10  LowerLimitDampingUnits=N*m/(deg/s)  LowerLimitTransitionRegionWidth=0.1  LowerLimitTransitionRegionWidthUnits=deg  UpperLimitSpecify=on  UpperLimitBound=1.047197551196598  UpperLimitBoundUnits=rad  UpperLimitStiffness=1e4  UpperLimitStiffnessUnits=N*m/deg  UpperLimitDamping=10  UpperLimitDampingUnits=N*m/(deg/s)  UpperLimitTransitionRegionWidth=0.1  UpperLimitTransitionRegionWidthUnits=deg  TorqueActuationMode=InputTorque  MotionActuationMode=ComputedMotion  SensePosition=on  SenseVelocity=on  SenseAcceleration=off  SenseTorqueForce=off  SenseLowerLimitTorqueForce=off  SenseUpperLimitTorqueForce=off
  waist_yaw1 : Subsystem
  wires:
  [qr_L_ankle_pitch] -> S_L_ankle_pitch/1
  cq_L_ankle_pitch/1 -> S_L_ankle_pitch/2
  S_L_ankle_pitch/1 -> K_L_ankle_pitch/1
  cw_L_ankle_pitch/1 -> B_L_ankle_pitch/1
  K_L_ankle_pitch/1 -> T_L_ankle_pitch/1
  B_L_ankle_pitch/1 -> T_L_ankle_pitch/2
  T_L_ankle_pitch/1 -> ct_L_ankle_pitch/1
  [qr_L_arm_twist] -> S_L_arm_twist/1
  cq_L_arm_twist/1 -> S_L_arm_twist/2
  S_L_arm_twist/1 -> K_L_arm_twist/1
  cw_L_arm_twist/1 -> B_L_arm_twist/1
  K_L_arm_twist/1 -> T_L_arm_twist/1
  B_L_arm_twist/1 -> T_L_arm_twist/2
  T_L_arm_twist/1 -> ct_L_arm_twist/1
  [qr_L_foot] -> S_L_foot/1
  cq_L_foot/1 -> S_L_foot/2
  S_L_foot/1 -> K_L_foot/1
  cw_L_foot/1 -> B_L_foot/1
  K_L_foot/1 -> T_L_foot/1
  B_L_foot/1 -> T_L_foot/2
  T_L_foot/1 -> ct_L_foot/1
  [qr_L_forearm] -> S_L_forearm/1
  cq_L_forearm/1 -> S_L_forearm/2
  S_L_forearm/1 -> K_L_forearm/1
  cw_L_forearm/1 -> B_L_forearm/1
  K_L_forearm/1 -> T_L_forearm/1
  B_L_forearm/1 -> T_L_forearm/2
  T_L_forearm/1 -> ct_L_forearm/1
  [qr_L_forearm_twist] -> S_L_forearm_twist/1
  cq_L_forearm_twist/1 -> S_L_forearm_twist/2
  S_L_forearm_twist/1 -> K_L_forearm_twist/1
  cw_L_forearm_twist/1 -> B_L_forearm_twist/1
  K_L_forearm_twist/1 -> T_L_forearm_twist/1
  B_L_forearm_twist/1 -> T_L_forearm_twist/2
  T_L_forearm_twist/1 -> ct_L_forearm_twist/1
  [qr_L_hand] -> S_L_hand/1
  cq_L_hand/1 -> S_L_hand/2
  S_L_hand/1 -> K_L_hand/1
  cw_L_hand/1 -> B_L_hand/1
  K_L_hand/1 -> T_L_hand/1
  B_L_hand/1 -> T_L_hand/2
  T_L_hand/1 -> ct_L_hand/1
  [qr_L_hip_aux] -> S_L_hip_aux/1
  cq_L_hip_aux/1 -> S_L_hip_aux/2
  S_L_hip_aux/1 -> K_L_hip_aux/1
  cw_L_hip_aux/1 -> B_L_hip_aux/1
  K_L_hip_aux/1 -> T_L_hip_aux/1
  B_L_hip_aux/1 -> T_L_hip_aux/2
  T_L_hip_aux/1 -> ct_L_hip_aux/1
  [qr_L_hip_roll] -> S_L_hip_roll/1
  cq_L_hip_roll/1 -> S_L_hip_roll/2
  S_L_hip_roll/1 -> K_L_hip_roll/1
  cw_L_hip_roll/1 -> B_L_hip_roll/1
  K_L_hip_roll/1 -> T_L_hip_roll/1
  B_L_hip_roll/1 -> T_L_hip_roll/2
  T_L_hip_roll/1 -> ct_L_hip_roll/1
  [qr_L_hip_yaw] -> S_L_hip_yaw/1
  cq_L_hip_yaw/1 -> S_L_hip_yaw/2
  S_L_hip_yaw/1 -> K_L_hip_yaw/1
  cw_L_hip_yaw/1 -> B_L_hip_yaw/1
  K_L_hip_yaw/1 -> T_L_hip_yaw/1
  B_L_hip_yaw/1 -> T_L_hip_yaw/2
  T_L_hip_yaw/1 -> ct_L_hip_yaw/1
  [qr_L_index1] -> S_L_index1/1
  cq_L_index1/1 -> S_L_index1/2
  S_L_index1/1 -> K_L_index1/1
  cw_L_index1/1 -> B_L_index1/1
  K_L_index1/1 -> T_L_index1/1
  B_L_index1/1 -> T_L_index1/2
  T_L_index1/1 -> ct_L_index1/1
  [qr_L_index2] -> S_L_index2/1
  cq_L_index2/1 -> S_L_index2/2
  S_L_index2/1 -> K_L_index2/1
  cw_L_index2/1 -> B_L_index2/1
  K_L_index2/1 -> T_L_index2/1
  B_L_index2/1 -> T_L_index2/2
  T_L_index2/1 -> ct_L_index2/1
  [qr_L_index3] -> S_L_index3/1
  cq_L_index3/1 -> S_L_index3/2
  S_L_index3/1 -> K_L_index3/1
  cw_L_index3/1 -> B_L_index3/1
  K_L_index3/1 -> T_L_index3/1
  B_L_index3/1 -> T_L_index3/2
  T_L_index3/1 -> ct_L_index3/1
  [qr_L_little1] -> S_L_little1/1
  cq_L_little1/1 -> S_L_little1/2
  S_L_little1/1 -> K_L_little1/1
  cw_L_little1/1 -> B_L_little1/1
  K_L_little1/1 -> T_L_little1/1
  B_L_little1/1 -> T_L_little1/2
  T_L_little1/1 -> ct_L_little1/1
  [qr_L_little2] -> S_L_little2/1
  cq_L_little2/1 -> S_L_little2/2
  S_L_little2/1 -> K_L_little2/1
  cw_L_little2/1 -> B_L_little2/1
  K_L_little2/1 -> T_L_little2/1
  B_L_little2/1 -> T_L_little2/2
  T_L_little2/1 -> ct_L_little2/1
  [qr_L_little3] -> S_L_little3/1
  cq_L_little3/1 -> S_L_little3/2
  S_L_little3/1 -> K_L_little3/1
  cw_L_little3/1 -> B_L_little3/1
  K_L_little3/1 -> T_L_little3/1
  B_L_little3/1 -> T_L_little3/2
  T_L_little3/1 -> ct_L_little3/1
  [qr_L_middle1] -> S_L_middle1/1
  cq_L_middle1/1 -> S_L_middle1/2
  S_L_middle1/1 -> K_L_middle1/1
  cw_L_middle1/1 -> B_L_middle1/1
  K_L_middle1/1 -> T_L_middle1/1
  B_L_middle1/1 -> T_L_middle1/2
  T_L_middle1/1 -> ct_L_middle1/1
  [qr_L_middle2] -> S_L_middle2/1
  cq_L_middle2/1 -> S_L_middle2/2
  S_L_middle2/1 -> K_L_middle2/1
  cw_L_middle2/1 -> B_L_middle2/1
  K_L_middle2/1 -> T_L_middle2/1
  B_L_middle2/1 -> T_L_middle2/2
  T_L_middle2/1 -> ct_L_middle2/1
  [qr_L_middle3] -> S_L_middle3/1
  cq_L_middle3/1 -> S_L_middle3/2
  S_L_middle3/1 -> K_L_middle3/1
  cw_L_middle3/1 -> B_L_middle3/1
  K_L_middle3/1 -> T_L_middle3/1
  B_L_middle3/1 -> T_L_middle3/2
  T_L_middle3/1 -> ct_L_middle3/1
  [qr_L_ring1] -> S_L_ring1/1
  cq_L_ring1/1 -> S_L_ring1/2
  S_L_ring1/1 -> K_L_ring1/1
  cw_L_ring1/1 -> B_L_ring1/1
  K_L_ring1/1 -> T_L_ring1/1
  B_L_ring1/1 -> T_L_ring1/2
  T_L_ring1/1 -> ct_L_ring1/1
  [qr_L_ring2] -> S_L_ring2/1
  cq_L_ring2/1 -> S_L_ring2/2
  S_L_ring2/1 -> K_L_ring2/1
  cw_L_ring2/1 -> B_L_ring2/1
  K_L_ring2/1 -> T_L_ring2/1
  B_L_ring2/1 -> T_L_ring2/2
  T_L_ring2/1 -> ct_L_ring2/1
  [qr_L_ring3] -> S_L_ring3/1
  cq_L_ring3/1 -> S_L_ring3/2
  S_L_ring3/1 -> K_L_ring3/1
  cw_L_ring3/1 -> B_L_ring3/1
  K_L_ring3/1 -> T_L_ring3/1
  B_L_ring3/1 -> T_L_ring3/2
  T_L_ring3/1 -> ct_L_ring3/1
  [qr_L_scapula] -> S_L_scapula/1
  cq_L_scapula/1 -> S_L_scapula/2
  S_L_scapula/1 -> K_L_scapula/1
  cw_L_scapula/1 -> B_L_scapula/1
  K_L_scapula/1 -> T_L_scapula/1
  B_L_scapula/1 -> T_L_scapula/2
  T_L_scapula/1 -> ct_L_scapula/1
  [qr_L_shin] -> S_L_shin/1
  cq_L_shin/1 -> S_L_shin/2
  S_L_shin/1 -> K_L_shin/1
  cw_L_shin/1 -> B_L_shin/1
  K_L_shin/1 -> T_L_shin/1
  B_L_shin/1 -> T_L_shin/2
  T_L_shin/1 -> ct_L_shin/1
  [qr_L_shoulder_roll] -> S_L_shoulder_roll/1
  cq_L_shoulder_roll/1 -> S_L_shoulder_roll/2
  S_L_shoulder_roll/1 -> K_L_shoulder_roll/1
  cw_L_shoulder_roll/1 -> B_L_shoulder_roll/1
  K_L_shoulder_roll/1 -> T_L_shoulder_roll/1
  B_L_shoulder_roll/1 -> T_L_shoulder_roll/2
  T_L_shoulder_roll/1 -> ct_L_shoulder_roll/1
  [qr_L_shoulder_yaw] -> S_L_shoulder_yaw/1
  cq_L_shoulder_yaw/1 -> S_L_shoulder_yaw/2
  S_L_shoulder_yaw/1 -> K_L_shoulder_yaw/1
  cw_L_shoulder_yaw/1 -> B_L_shoulder_yaw/1
  K_L_shoulder_yaw/1 -> T_L_shoulder_yaw/1
  B_L_shoulder_yaw/1 -> T_L_shoulder_yaw/2
  T_L_shoulder_yaw/1 -> ct_L_shoulder_yaw/1
  [qr_L_thigh] -> S_L_thigh/1
  cq_L_thigh/1 -> S_L_thigh/2
  S_L_thigh/1 -> K_L_thigh/1
  cw_L_thigh/1 -> B_L_thigh/1
  K_L_thigh/1 -> T_L_thigh/1
  B_L_thigh/1 -> T_L_thigh/2
  T_L_thigh/1 -> ct_L_thigh/1
  [qr_L_thumb1] -> S_L_thumb1/1
  cq_L_thumb1/1 -> S_L_thumb1/2
  S_L_thumb1/1 -> K_L_thumb1/1
  cw_L_thumb1/1 -> B_L_thumb1/1
  K_L_thumb1/1 -> T_L_thumb1/1
  B_L_thumb1/1 -> T_L_thumb1/2
  T_L_thumb1/1 -> ct_L_thumb1/1
  [qr_L_thumb2] -> S_L_thumb2/1
  cq_L_thumb2/1 -> S_L_thumb2/2
  S_L_thumb2/1 -> K_L_thumb2/1
  cw_L_thumb2/1 -> B_L_thumb2/1
  K_L_thumb2/1 -> T_L_thumb2/1
  B_L_thumb2/1 -> T_L_thumb2/2
  T_L_thumb2/1 -> ct_L_thumb2/1
  [qr_L_thumb3] -> S_L_thumb3/1
  cq_L_thumb3/1 -> S_L_thumb3/2
  S_L_thumb3/1 -> K_L_thumb3/1
  cw_L_thumb3/1 -> B_L_thumb3/1
  K_L_thumb3/1 -> T_L_thumb3/1
  B_L_thumb3/1 -> T_L_thumb3/2
  T_L_thumb3/1 -> ct_L_thumb3/1
  [qr_L_toe] -> S_L_toe/1
  cq_L_toe/1 -> S_L_toe/2
  S_L_toe/1 -> K_L_toe/1
  cw_L_toe/1 -> B_L_toe/1
  K_L_toe/1 -> T_L_toe/1
  B_L_toe/1 -> T_L_toe/2
  T_L_toe/1 -> ct_L_toe/1
  [qr_L_upper_arm] -> S_L_upper_arm/1
  cq_L_upper_arm/1 -> S_L_upper_arm/2
  S_L_upper_arm/1 -> K_L_upper_arm/1
  cw_L_upper_arm/1 -> B_L_upper_arm/1
  K_L_upper_arm/1 -> T_L_upper_arm/1
  B_L_upper_arm/1 -> T_L_upper_arm/2
  T_L_upper_arm/1 -> ct_L_upper_arm/1
  [qr_L_wrist_roll] -> S_L_wrist_roll/1
  cq_L_wrist_roll/1 -> S_L_wrist_roll/2
  S_L_wrist_roll/1 -> K_L_wrist_roll/1
  cw_L_wrist_roll/1 -> B_L_wrist_roll/1
  K_L_wrist_roll/1 -> T_L_wrist_roll/1
  B_L_wrist_roll/1 -> T_L_wrist_roll/2
  T_L_wrist_roll/1 -> ct_L_wrist_roll/1
  [qr_L_wrist_yaw] -> S_L_wrist_yaw/1
  cq_L_wrist_yaw/1 -> S_L_wrist_yaw/2
  S_L_wrist_yaw/1 -> K_L_wrist_yaw/1
  cw_L_wrist_yaw/1 -> B_L_wrist_yaw/1
  K_L_wrist_yaw/1 -> T_L_wrist_yaw/1
  B_L_wrist_yaw/1 -> T_L_wrist_yaw/2
  T_L_wrist_yaw/1 -> ct_L_wrist_yaw/1
  [qr_R_ankle_pitch] -> S_R_ankle_pitch/1
  cq_R_ankle_pitch/1 -> S_R_ankle_pitch/2
  S_R_ankle_pitch/1 -> K_R_ankle_pitch/1
  cw_R_ankle_pitch/1 -> B_R_ankle_pitch/1
  K_R_ankle_pitch/1 -> T_R_ankle_pitch/1
  B_R_ankle_pitch/1 -> T_R_ankle_pitch/2
  T_R_ankle_pitch/1 -> ct_R_ankle_pitch/1
  [qr_R_arm_twist] -> S_R_arm_twist/1
  cq_R_arm_twist/1 -> S_R_arm_twist/2
  S_R_arm_twist/1 -> K_R_arm_twist/1
  cw_R_arm_twist/1 -> B_R_arm_twist/1
  K_R_arm_twist/1 -> T_R_arm_twist/1
  B_R_arm_twist/1 -> T_R_arm_twist/2
  T_R_arm_twist/1 -> ct_R_arm_twist/1
  [qr_R_foot] -> S_R_foot/1
  cq_R_foot/1 -> S_R_foot/2
  S_R_foot/1 -> K_R_foot/1
  cw_R_foot/1 -> B_R_foot/1
  K_R_foot/1 -> T_R_foot/1
  B_R_foot/1 -> T_R_foot/2
  T_R_foot/1 -> ct_R_foot/1
  [qr_R_forearm] -> S_R_forearm/1
  cq_R_forearm/1 -> S_R_forearm/2
  S_R_forearm/1 -> K_R_forearm/1
  cw_R_forearm/1 -> B_R_forearm/1
  K_R_forearm/1 -> T_R_forearm/1
  B_R_forearm/1 -> T_R_forearm/2
  T_R_forearm/1 -> ct_R_forearm/1
  [qr_R_forearm_twist] -> S_R_forearm_twist/1
  cq_R_forearm_twist/1 -> S_R_forearm_twist/2
  S_R_forearm_twist/1 -> K_R_forearm_twist/1
  cw_R_forearm_twist/1 -> B_R_forearm_twist/1
  K_R_forearm_twist/1 -> T_R_forearm_twist/1
  B_R_forearm_twist/1 -> T_R_forearm_twist/2
  T_R_forearm_twist/1 -> ct_R_forearm_twist/1
  [qr_R_hand] -> S_R_hand/1
  cq_R_hand/1 -> S_R_hand/2
  S_R_hand/1 -> K_R_hand/1
  cw_R_hand/1 -> B_R_hand/1
  K_R_hand/1 -> T_R_hand/1
  B_R_hand/1 -> T_R_hand/2
  T_R_hand/1 -> ct_R_hand/1
  [qr_R_hip_aux] -> S_R_hip_aux/1
  cq_R_hip_aux/1 -> S_R_hip_aux/2
  S_R_hip_aux/1 -> K_R_hip_aux/1
  cw_R_hip_aux/1 -> B_R_hip_aux/1
  K_R_hip_aux/1 -> T_R_hip_aux/1
  B_R_hip_aux/1 -> T_R_hip_aux/2
  T_R_hip_aux/1 -> ct_R_hip_aux/1
  [qr_R_hip_roll] -> S_R_hip_roll/1
  cq_R_hip_roll/1 -> S_R_hip_roll/2
  S_R_hip_roll/1 -> K_R_hip_roll/1
  cw_R_hip_roll/1 -> B_R_hip_roll/1
  K_R_hip_roll/1 -> T_R_hip_roll/1
  B_R_hip_roll/1 -> T_R_hip_roll/2
  T_R_hip_roll/1 -> ct_R_hip_roll/1
  [qr_R_hip_yaw] -> S_R_hip_yaw/1
  cq_R_hip_yaw/1 -> S_R_hip_yaw/2
  S_R_hip_yaw/1 -> K_R_hip_yaw/1
  cw_R_hip_yaw/1 -> B_R_hip_yaw/1
  K_R_hip_yaw/1 -> T_R_hip_yaw/1
  B_R_hip_yaw/1 -> T_R_hip_yaw/2
  T_R_hip_yaw/1 -> ct_R_hip_yaw/1
  [qr_R_index1] -> S_R_index1/1
  cq_R_index1/1 -> S_R_index1/2
  S_R_index1/1 -> K_R_index1/1
  cw_R_index1/1 -> B_R_index1/1
  K_R_index1/1 -> T_R_index1/1
  B_R_index1/1 -> T_R_index1/2
  T_R_index1/1 -> ct_R_index1/1
  [qr_R_index2] -> S_R_index2/1
  cq_R_index2/1 -> S_R_index2/2
  S_R_index2/1 -> K_R_index2/1
  cw_R_index2/1 -> B_R_index2/1
  K_R_index2/1 -> T_R_index2/1
  B_R_index2/1 -> T_R_index2/2
  T_R_index2/1 -> ct_R_index2/1
  [qr_R_index3] -> S_R_index3/1
  cq_R_index3/1 -> S_R_index3/2
  S_R_index3/1 -> K_R_index3/1
  cw_R_index3/1 -> B_R_index3/1
  K_R_index3/1 -> T_R_index3/1
  B_R_index3/1 -> T_R_index3/2
  T_R_index3/1 -> ct_R_index3/1
  [qr_R_little1] -> S_R_little1/1
  cq_R_little1/1 -> S_R_little1/2
  S_R_little1/1 -> K_R_little1/1
  cw_R_little1/1 -> B_R_little1/1
  K_R_little1/1 -> T_R_little1/1
  B_R_little1/1 -> T_R_little1/2
  T_R_little1/1 -> ct_R_little1/1
  [qr_R_little2] -> S_R_little2/1
  cq_R_little2/1 -> S_R_little2/2
  S_R_little2/1 -> K_R_little2/1
  cw_R_little2/1 -> B_R_little2/1
  K_R_little2/1 -> T_R_little2/1
  B_R_little2/1 -> T_R_little2/2
  T_R_little2/1 -> ct_R_little2/1
  [qr_R_little3] -> S_R_little3/1
  cq_R_little3/1 -> S_R_little3/2
  S_R_little3/1 -> K_R_little3/1
  cw_R_little3/1 -> B_R_little3/1
  K_R_little3/1 -> T_R_little3/1
  B_R_little3/1 -> T_R_little3/2
  T_R_little3/1 -> ct_R_little3/1
  [qr_R_middle1] -> S_R_middle1/1
  cq_R_middle1/1 -> S_R_middle1/2
  S_R_middle1/1 -> K_R_middle1/1
  cw_R_middle1/1 -> B_R_middle1/1
  K_R_middle1/1 -> T_R_middle1/1
  B_R_middle1/1 -> T_R_middle1/2
  T_R_middle1/1 -> ct_R_middle1/1
  [qr_R_middle2] -> S_R_middle2/1
  cq_R_middle2/1 -> S_R_middle2/2
  S_R_middle2/1 -> K_R_middle2/1
  cw_R_middle2/1 -> B_R_middle2/1
  K_R_middle2/1 -> T_R_middle2/1
  B_R_middle2/1 -> T_R_middle2/2
  T_R_middle2/1 -> ct_R_middle2/1
  [qr_R_middle3] -> S_R_middle3/1
  cq_R_middle3/1 -> S_R_middle3/2
  S_R_middle3/1 -> K_R_middle3/1
  cw_R_middle3/1 -> B_R_middle3/1
  K_R_middle3/1 -> T_R_middle3/1
  B_R_middle3/1 -> T_R_middle3/2
  T_R_middle3/1 -> ct_R_middle3/1
  [qr_R_ring1] -> S_R_ring1/1
  cq_R_ring1/1 -> S_R_ring1/2
  S_R_ring1/1 -> K_R_ring1/1
  cw_R_ring1/1 -> B_R_ring1/1
  K_R_ring1/1 -> T_R_ring1/1
  B_R_ring1/1 -> T_R_ring1/2
  T_R_ring1/1 -> ct_R_ring1/1
  [qr_R_ring2] -> S_R_ring2/1
  cq_R_ring2/1 -> S_R_ring2/2
  S_R_ring2/1 -> K_R_ring2/1
  cw_R_ring2/1 -> B_R_ring2/1
  K_R_ring2/1 -> T_R_ring2/1
  B_R_ring2/1 -> T_R_ring2/2
  T_R_ring2/1 -> ct_R_ring2/1
  [qr_R_ring3] -> S_R_ring3/1
  cq_R_ring3/1 -> S_R_ring3/2
  S_R_ring3/1 -> K_R_ring3/1
  cw_R_ring3/1 -> B_R_ring3/1
  K_R_ring3/1 -> T_R_ring3/1
  B_R_ring3/1 -> T_R_ring3/2
  T_R_ring3/1 -> ct_R_ring3/1
  [qr_R_scapula] -> S_R_scapula/1
  cq_R_scapula/1 -> S_R_scapula/2
  S_R_scapula/1 -> K_R_scapula/1
  cw_R_scapula/1 -> B_R_scapula/1
  K_R_scapula/1 -> T_R_scapula/1
  B_R_scapula/1 -> T_R_scapula/2
  T_R_scapula/1 -> ct_R_scapula/1
  [qr_R_shin] -> S_R_shin/1
  cq_R_shin/1 -> S_R_shin/2
  S_R_shin/1 -> K_R_shin/1
  cw_R_shin/1 -> B_R_shin/1
  K_R_shin/1 -> T_R_shin/1
  B_R_shin/1 -> T_R_shin/2
  T_R_shin/1 -> ct_R_shin/1
  [qr_R_shoulder_roll] -> S_R_shoulder_roll/1
  cq_R_shoulder_roll/1 -> S_R_shoulder_roll/2
  S_R_shoulder_roll/1 -> K_R_shoulder_roll/1
  cw_R_shoulder_roll/1 -> B_R_shoulder_roll/1
  K_R_shoulder_roll/1 -> T_R_shoulder_roll/1
  B_R_shoulder_roll/1 -> T_R_shoulder_roll/2
  T_R_shoulder_roll/1 -> ct_R_shoulder_roll/1
  [qr_R_shoulder_yaw] -> S_R_shoulder_yaw/1
  cq_R_shoulder_yaw/1 -> S_R_shoulder_yaw/2
  S_R_shoulder_yaw/1 -> K_R_shoulder_yaw/1
  cw_R_shoulder_yaw/1 -> B_R_shoulder_yaw/1
  K_R_shoulder_yaw/1 -> T_R_shoulder_yaw/1
  B_R_shoulder_yaw/1 -> T_R_shoulder_yaw/2
  T_R_shoulder_yaw/1 -> ct_R_shoulder_yaw/1
  [qr_R_thigh] -> S_R_thigh/1
  cq_R_thigh/1 -> S_R_thigh/2
  S_R_thigh/1 -> K_R_thigh/1
  cw_R_thigh/1 -> B_R_thigh/1
  K_R_thigh/1 -> T_R_thigh/1
  B_R_thigh/1 -> T_R_thigh/2
  T_R_thigh/1 -> ct_R_thigh/1
  [qr_R_thumb1] -> S_R_thumb1/1
  cq_R_thumb1/1 -> S_R_thumb1/2
  S_R_thumb1/1 -> K_R_thumb1/1
  cw_R_thumb1/1 -> B_R_thumb1/1
  K_R_thumb1/1 -> T_R_thumb1/1
  B_R_thumb1/1 -> T_R_thumb1/2
  T_R_thumb1/1 -> ct_R_thumb1/1
  [qr_R_thumb2] -> S_R_thumb2/1
  cq_R_thumb2/1 -> S_R_thumb2/2
  S_R_thumb2/1 -> K_R_thumb2/1
  cw_R_thumb2/1 -> B_R_thumb2/1
  K_R_thumb2/1 -> T_R_thumb2/1
  B_R_thumb2/1 -> T_R_thumb2/2
  T_R_thumb2/1 -> ct_R_thumb2/1
  [qr_R_thumb3] -> S_R_thumb3/1
  cq_R_thumb3/1 -> S_R_thumb3/2
  S_R_thumb3/1 -> K_R_thumb3/1
  cw_R_thumb3/1 -> B_R_thumb3/1
  K_R_thumb3/1 -> T_R_thumb3/1
  B_R_thumb3/1 -> T_R_thumb3/2
  T_R_thumb3/1 -> ct_R_thumb3/1
  [qr_R_toe] -> S_R_toe/1
  cq_R_toe/1 -> S_R_toe/2
  S_R_toe/1 -> K_R_toe/1
  cw_R_toe/1 -> B_R_toe/1
  K_R_toe/1 -> T_R_toe/1
  B_R_toe/1 -> T_R_toe/2
  T_R_toe/1 -> ct_R_toe/1
  [qr_R_upper_arm] -> S_R_upper_arm/1
  cq_R_upper_arm/1 -> S_R_upper_arm/2
  S_R_upper_arm/1 -> K_R_upper_arm/1
  cw_R_upper_arm/1 -> B_R_upper_arm/1
  K_R_upper_arm/1 -> T_R_upper_arm/1
  B_R_upper_arm/1 -> T_R_upper_arm/2
  T_R_upper_arm/1 -> ct_R_upper_arm/1
  [qr_R_wrist_roll] -> S_R_wrist_roll/1
  cq_R_wrist_roll/1 -> S_R_wrist_roll/2
  S_R_wrist_roll/1 -> K_R_wrist_roll/1
  cw_R_wrist_roll/1 -> B_R_wrist_roll/1
  K_R_wrist_roll/1 -> T_R_wrist_roll/1
  B_R_wrist_roll/1 -> T_R_wrist_roll/2
  T_R_wrist_roll/1 -> ct_R_wrist_roll/1
  [qr_R_wrist_yaw] -> S_R_wrist_yaw/1
  cq_R_wrist_yaw/1 -> S_R_wrist_yaw/2
  S_R_wrist_yaw/1 -> K_R_wrist_yaw/1
  cw_R_wrist_yaw/1 -> B_R_wrist_yaw/1
  K_R_wrist_yaw/1 -> T_R_wrist_yaw/1
  B_R_wrist_yaw/1 -> T_R_wrist_yaw/2
  T_R_wrist_yaw/1 -> ct_R_wrist_yaw/1
  [qr_neck_pitch] -> S_neck_pitch/1
  cq_neck_pitch/1 -> S_neck_pitch/2
  S_neck_pitch/1 -> K_neck_pitch/1
  cw_neck_pitch/1 -> B_neck_pitch/1
  K_neck_pitch/1 -> T_neck_pitch/1
  B_neck_pitch/1 -> T_neck_pitch/2
  T_neck_pitch/1 -> ct_neck_pitch/1
  [qr_neck_roll] -> S_neck_roll/1
  cq_neck_roll/1 -> S_neck_roll/2
  S_neck_roll/1 -> K_neck_roll/1
  cw_neck_roll/1 -> B_neck_roll/1
  K_neck_roll/1 -> T_neck_roll/1
  B_neck_roll/1 -> T_neck_roll/2
  T_neck_roll/1 -> ct_neck_roll/1
  [qr_neck_yaw] -> S_neck_yaw/1
  cq_neck_yaw/1 -> S_neck_yaw/2
  S_neck_yaw/1 -> K_neck_yaw/1
  cw_neck_yaw/1 -> B_neck_yaw/1
  K_neck_yaw/1 -> T_neck_yaw/1
  B_neck_yaw/1 -> T_neck_yaw/2
  T_neck_yaw/1 -> ct_neck_yaw/1
  [qr_waist_pitch] -> S_waist_pitch/1
  cq_waist_pitch/1 -> S_waist_pitch/2
  S_waist_pitch/1 -> K_waist_pitch/1
  cw_waist_pitch/1 -> B_waist_pitch/1
  K_waist_pitch/1 -> T_waist_pitch/1
  B_waist_pitch/1 -> T_waist_pitch/2
  T_waist_pitch/1 -> ct_waist_pitch/1
  [qr_waist_roll] -> S_waist_roll/1
  cq_waist_roll/1 -> S_waist_roll/2
  S_waist_roll/1 -> K_waist_roll/1
  cw_waist_roll/1 -> B_waist_roll/1
  K_waist_roll/1 -> T_waist_roll/1
  B_waist_roll/1 -> T_waist_roll/2
  T_waist_roll/1 -> ct_waist_roll/1
  [qr_waist_yaw] -> S_waist_yaw/1
  cq_waist_yaw/1 -> S_waist_yaw/2
  S_waist_yaw/1 -> K_waist_yaw/1
  cw_waist_yaw/1 -> B_waist_yaw/1
  K_waist_yaw/1 -> T_waist_yaw/1
  B_waist_yaw/1 -> T_waist_yaw/2
  T_waist_yaw/1 -> ct_waist_yaw/1
  qref/1 -> qref_demux/1
  qref_demux/1 -> [qr_L_ankle_pitch]
  qref_demux/2 -> [qr_L_arm_twist]
  qref_demux/3 -> [qr_L_foot]
  qref_demux/4 -> [qr_L_forearm]
  qref_demux/5 -> [qr_L_forearm_twist]
  qref_demux/6 -> [qr_L_hand]
  qref_demux/7 -> [qr_L_hip_aux]
  qref_demux/8 -> [qr_L_hip_roll]
  qref_demux/9 -> [qr_L_hip_yaw]
  qref_demux/10 -> [qr_L_index1]
  qref_demux/11 -> [qr_L_index2]
  qref_demux/12 -> [qr_L_index3]
  qref_demux/13 -> [qr_L_little1]
  qref_demux/14 -> [qr_L_little2]
  qref_demux/15 -> [qr_L_little3]
  qref_demux/16 -> [qr_L_middle1]
  qref_demux/17 -> [qr_L_middle2]
  qref_demux/18 -> [qr_L_middle3]
  qref_demux/19 -> [qr_L_ring1]
  qref_demux/20 -> [qr_L_ring2]
  qref_demux/21 -> [qr_L_ring3]
  qref_demux/22 -> [qr_L_scapula]
  qref_demux/23 -> [qr_L_shin]
  qref_demux/24 -> [qr_L_shoulder_roll]
  qref_demux/25 -> [qr_L_shoulder_yaw]
  qref_demux/26 -> [qr_L_thigh]
  qref_demux/27 -> [qr_L_thumb1]
  qref_demux/28 -> [qr_L_thumb2]
  qref_demux/29 -> [qr_L_thumb3]
  qref_demux/30 -> [qr_L_toe]
  qref_demux/31 -> [qr_L_upper_arm]
  qref_demux/32 -> [qr_L_wrist_roll]
  qref_demux/33 -> [qr_L_wrist_yaw]
  qref_demux/34 -> [qr_R_ankle_pitch]
  qref_demux/35 -> [qr_R_arm_twist]
  qref_demux/36 -> [qr_R_foot]
  qref_demux/37 -> [qr_R_forearm]
  qref_demux/38 -> [qr_R_forearm_twist]
  qref_demux/39 -> [qr_R_hand]
  qref_demux/40 -> [qr_R_hip_aux]
  qref_demux/41 -> [qr_R_hip_roll]
  qref_demux/42 -> [qr_R_hip_yaw]
  qref_demux/43 -> [qr_R_index1]
  qref_demux/44 -> [qr_R_index2]
  qref_demux/45 -> [qr_R_index3]
  qref_demux/46 -> [qr_R_little1]
  qref_demux/47 -> [qr_R_little2]
  qref_demux/48 -> [qr_R_little3]
  qref_demux/49 -> [qr_R_middle1]
  qref_demux/50 -> [qr_R_middle2]
  qref_demux/51 -> [qr_R_middle3]
  qref_demux/52 -> [qr_R_ring1]
  qref_demux/53 -> [qr_R_ring2]
  qref_demux/54 -> [qr_R_ring3]
  qref_demux/55 -> [qr_R_scapula]
  qref_demux/56 -> [qr_R_shin]
  qref_demux/57 -> [qr_R_shoulder_roll]
  qref_demux/58 -> [qr_R_shoulder_yaw]
  qref_demux/59 -> [qr_R_thigh]
  qref_demux/60 -> [qr_R_thumb1]
  qref_demux/61 -> [qr_R_thumb2]
  qref_demux/62 -> [qr_R_thumb3]
  qref_demux/63 -> [qr_R_toe]
  qref_demux/64 -> [qr_R_upper_arm]
  qref_demux/65 -> [qr_R_wrist_roll]
  qref_demux/66 -> [qr_R_wrist_yaw]
  qref_demux/67 -> [qr_neck_pitch]
  qref_demux/68 -> [qr_neck_roll]
  qref_demux/69 -> [qr_neck_yaw]
  qref_demux/70 -> [qr_waist_pitch]
  qref_demux/71 -> [qr_waist_roll]
  qref_demux/72 -> [qr_waist_yaw]
  connections:
  L_ankle_pitch/RConn1 -- L_ankle_pitch1/LConn1
  L_ankle_pitch1/RConn1 -- L_foot/LConn1
  L_hand/RConn1 -- L_hand1/LConn1
  R_middle3/RConn1 -- R_middle6/LConn1
  R_ring1/RConn1 -- R_ring4/LConn1
  R_ring2/LConn1 -- R_ring4/RConn1
  R_ring2/RConn1 -- R_ring5/LConn1
  R_ring3/LConn1 -- R_ring5/RConn1
  R_ring3/RConn1 -- R_ring6/LConn1
  R_scapula/RConn1 -- R_scapula1/LConn1
  R_scapula1/RConn1 -- R_shoulder_yaw/LConn1
  R_shin/RConn1 -- R_shin1/LConn1
  R_ankle_pitch/LConn1 -- R_shin1/RConn1
  L_hand1/RConn5 -- L_index1/LConn1
  R_shoulder_roll/RConn1 -- R_shoulder_roll1/LConn1
  R_shoulder_roll1/RConn1 -- R_upper_arm/LConn1
  R_shoulder_yaw/RConn1 -- R_shoulder_yaw1/LConn1
  R_shoulder_roll/LConn1 -- R_shoulder_yaw1/RConn1
  R_thigh/RConn1 -- R_thigh1/LConn1
  R_shin/LConn1 -- R_thigh1/RConn1
  R_thumb1/RConn1 -- R_thumb4/LConn1
  R_thumb2/LConn1 -- R_thumb4/RConn1
  R_thumb2/RConn1 -- R_thumb5/LConn1
  R_thumb3/LConn1 -- R_thumb5/RConn1
  L_hand1/RConn4 -- L_little1/LConn1
  R_thumb3/RConn1 -- R_thumb6/LConn1
  R_toe/RConn1 -- R_toe1/LConn1
  R_upper_arm/RConn1 -- R_upper_arm1/LConn1
  R_arm_twist/LConn1 -- R_upper_arm1/RConn1
  R_wrist_roll/RConn1 -- R_wrist_roll1/LConn1
  R_hand/LConn1 -- R_wrist_roll1/RConn1
  R_wrist_yaw/RConn1 -- R_wrist_yaw1/LConn1
  R_wrist_roll/LConn1 -- R_wrist_yaw1/RConn1
  head/LConn1 -- neck_pitch/RConn1
  neck_roll/RConn1 -- neck_roll1/LConn1
  L_hand1/RConn3 -- L_middle1/LConn1
  neck_pitch/LConn1 -- neck_roll1/RConn1
  neck_yaw/RConn1 -- neck_yaw1/LConn1
  neck_roll/LConn1 -- neck_yaw1/RConn1
  L_hip_aux/LConn1 -- pelvis/RConn3
  R_hip_aux/LConn1 -- pelvis/RConn2
  pelvis/RConn1 -- waist_yaw/LConn1
  torso/LConn1 -- waist_pitch/RConn1
  L_scapula/LConn1 -- torso/RConn3
  R_scapula/LConn1 -- torso/RConn2
  neck_yaw/LConn1 -- torso/RConn1
  L_hand1/RConn2 -- L_ring1/LConn1
  waist_roll/RConn1 -- waist_roll1/LConn1
  waist_pitch/LConn1 -- waist_roll1/RConn1
  waist_yaw/RConn1 -- waist_yaw1/LConn1
  waist_roll/LConn1 -- waist_yaw1/RConn1
  World/RConn1 -- MechanismConfiguration/RConn1 -- Solver Configuration/RConn1 -- pelvis/LConn1
  L_hand1/RConn1 -- L_thumb1/LConn1
  L_hip_aux/RConn1 -- L_hip_aux1/LConn1
  L_hip_aux1/RConn1 -- L_hip_yaw/LConn1
  L_hip_roll/RConn1 -- L_hip_roll1/LConn1
  L_hip_roll1/RConn1 -- L_thigh/LConn1
  L_arm_twist/RConn1 -- L_arm_twist1/LConn1
  L_hip_yaw/RConn1 -- L_hip_yaw1/LConn1
  L_hip_roll/LConn1 -- L_hip_yaw1/RConn1
  L_index1/RConn1 -- L_index4/LConn1
  L_index2/LConn1 -- L_index4/RConn1
  L_index2/RConn1 -- L_index5/LConn1
  L_index3/LConn1 -- L_index5/RConn1
  L_index3/RConn1 -- L_index6/LConn1
  L_little1/RConn1 -- L_little4/LConn1
  L_little2/LConn1 -- L_little4/RConn1
  L_little2/RConn1 -- L_little5/LConn1
  L_arm_twist1/RConn1 -- L_forearm/LConn1
  L_little3/LConn1 -- L_little5/RConn1
  L_little3/RConn1 -- L_little6/LConn1
  L_middle1/RConn1 -- L_middle4/LConn1
  L_middle2/LConn1 -- L_middle4/RConn1
  L_middle2/RConn1 -- L_middle5/LConn1
  L_middle3/LConn1 -- L_middle5/RConn1
  L_middle3/RConn1 -- L_middle6/LConn1
  L_ring1/RConn1 -- L_ring4/LConn1
  L_ring2/LConn1 -- L_ring4/RConn1
  L_ring2/RConn1 -- L_ring5/LConn1
  L_foot/RConn1 -- L_foot1/LConn1
  L_ring3/LConn1 -- L_ring5/RConn1
  L_ring3/RConn1 -- L_ring6/LConn1
  L_scapula/RConn1 -- L_scapula1/LConn1
  L_scapula1/RConn1 -- L_shoulder_yaw/LConn1
  L_shin/RConn1 -- L_shin1/LConn1
  L_ankle_pitch/LConn1 -- L_shin1/RConn1
  L_shoulder_roll/RConn1 -- L_shoulder_roll1/LConn1
  L_shoulder_roll1/RConn1 -- L_upper_arm/LConn1
  L_shoulder_yaw/RConn1 -- L_shoulder_yaw1/LConn1
  L_shoulder_roll/LConn1 -- L_shoulder_yaw1/RConn1
  L_foot1/RConn1 -- L_toe/LConn1
  L_thigh/RConn1 -- L_thigh1/LConn1
  L_shin/LConn1 -- L_thigh1/RConn1
  L_thumb1/RConn1 -- L_thumb4/LConn1
  L_thumb2/LConn1 -- L_thumb4/RConn1
  L_thumb2/RConn1 -- L_thumb5/LConn1
  L_thumb3/LConn1 -- L_thumb5/RConn1
  L_thumb3/RConn1 -- L_thumb6/LConn1
  L_toe/RConn1 -- L_toe1/LConn1
  L_upper_arm/RConn1 -- L_upper_arm1/LConn1
  L_arm_twist/LConn1 -- L_upper_arm1/RConn1
  L_forearm/RConn1 -- L_forearm1/LConn1
  L_wrist_roll/RConn1 -- L_wrist_roll1/LConn1
  L_hand/LConn1 -- L_wrist_roll1/RConn1
  L_wrist_yaw/RConn1 -- L_wrist_yaw1/LConn1
  L_wrist_roll/LConn1 -- L_wrist_yaw1/RConn1
  R_ankle_pitch/RConn1 -- R_ankle_pitch1/LConn1
  R_ankle_pitch1/RConn1 -- R_foot/LConn1
  R_arm_twist/RConn1 -- R_arm_twist1/LConn1
  R_arm_twist1/RConn1 -- R_forearm/LConn1
  R_foot/RConn1 -- R_foot1/LConn1
  R_foot1/RConn1 -- R_toe/LConn1
  L_forearm1/RConn1 -- L_forearm_twist/LConn1
  R_forearm/RConn1 -- R_forearm1/LConn1
  R_forearm1/RConn1 -- R_forearm_twist/LConn1
  R_forearm_twist/RConn1 -- R_forearm_twist1/LConn1
  R_forearm_twist1/RConn1 -- R_wrist_yaw/LConn1
  R_hand/RConn1 -- R_hand1/LConn1
  R_hand1/RConn5 -- R_index1/LConn1
  R_hand1/RConn4 -- R_little1/LConn1
  R_hand1/RConn3 -- R_middle1/LConn1
  R_hand1/RConn2 -- R_ring1/LConn1
  R_hand1/RConn1 -- R_thumb1/LConn1
  L_forearm_twist/RConn1 -- L_forearm_twist1/LConn1
  R_hip_aux/RConn1 -- R_hip_aux1/LConn1
  R_hip_aux1/RConn1 -- R_hip_yaw/LConn1
  R_hip_roll/RConn1 -- R_hip_roll1/LConn1
  R_hip_roll1/RConn1 -- R_thigh/LConn1
  R_hip_yaw/RConn1 -- R_hip_yaw1/LConn1
  R_hip_roll/LConn1 -- R_hip_yaw1/RConn1
  R_index1/RConn1 -- R_index4/LConn1
  R_index2/LConn1 -- R_index4/RConn1
  R_index2/RConn1 -- R_index5/LConn1
  R_index3/LConn1 -- R_index5/RConn1
  L_forearm_twist1/RConn1 -- L_wrist_yaw/LConn1
  R_index3/RConn1 -- R_index6/LConn1
  R_little1/RConn1 -- R_little4/LConn1
  R_little2/LConn1 -- R_little4/RConn1
  R_little2/RConn1 -- R_little5/LConn1
  R_little3/LConn1 -- R_little5/RConn1
  R_little3/RConn1 -- R_little6/LConn1
  R_middle1/RConn1 -- R_middle4/LConn1
  R_middle2/LConn1 -- R_middle4/RConn1
  R_middle2/RConn1 -- R_middle5/LConn1
  R_middle3/LConn1 -- R_middle5/RConn1
  L_ankle_pitch/RConn2 -- cq_L_ankle_pitch/LConn1
  L_ankle_pitch/RConn3 -- cw_L_ankle_pitch/LConn1
  ct_L_ankle_pitch/RConn1 -- L_ankle_pitch/LConn2
  L_arm_twist/RConn2 -- cq_L_arm_twist/LConn1
  L_arm_twist/RConn3 -- cw_L_arm_twist/LConn1
  ct_L_arm_twist/RConn1 -- L_arm_twist/LConn2
  L_foot/RConn2 -- cq_L_foot/LConn1
  L_foot/RConn3 -- cw_L_foot/LConn1
  ct_L_foot/RConn1 -- L_foot/LConn2
  L_forearm/RConn2 -- cq_L_forearm/LConn1
  L_forearm/RConn3 -- cw_L_forearm/LConn1
  ct_L_forearm/RConn1 -- L_forearm/LConn2
  L_forearm_twist/RConn2 -- cq_L_forearm_twist/LConn1
  L_forearm_twist/RConn3 -- cw_L_forearm_twist/LConn1
  ct_L_forearm_twist/RConn1 -- L_forearm_twist/LConn2
  L_hand/RConn2 -- cq_L_hand/LConn1
  L_hand/RConn3 -- cw_L_hand/LConn1
  ct_L_hand/RConn1 -- L_hand/LConn2
  L_hip_aux/RConn2 -- cq_L_hip_aux/LConn1
  L_hip_aux/RConn3 -- cw_L_hip_aux/LConn1
  ct_L_hip_aux/RConn1 -- L_hip_aux/LConn2
  L_hip_roll/RConn2 -- cq_L_hip_roll/LConn1
  L_hip_roll/RConn3 -- cw_L_hip_roll/LConn1
  ct_L_hip_roll/RConn1 -- L_hip_roll/LConn2
  L_hip_yaw/RConn2 -- cq_L_hip_yaw/LConn1
  L_hip_yaw/RConn3 -- cw_L_hip_yaw/LConn1
  ct_L_hip_yaw/RConn1 -- L_hip_yaw/LConn2
  L_index1/RConn2 -- cq_L_index1/LConn1
  L_index1/RConn3 -- cw_L_index1/LConn1
  ct_L_index1/RConn1 -- L_index1/LConn2
  L_index2/RConn2 -- cq_L_index2/LConn1
  L_index2/RConn3 -- cw_L_index2/LConn1
  ct_L_index2/RConn1 -- L_index2/LConn2
  L_index3/RConn2 -- cq_L_index3/LConn1
  L_index3/RConn3 -- cw_L_index3/LConn1
  ct_L_index3/RConn1 -- L_index3/LConn2
  L_little1/RConn2 -- cq_L_little1/LConn1
  L_little1/RConn3 -- cw_L_little1/LConn1
  ct_L_little1/RConn1 -- L_little1/LConn2
  L_little2/RConn2 -- cq_L_little2/LConn1
  L_little2/RConn3 -- cw_L_little2/LConn1
  ct_L_little2/RConn1 -- L_little2/LConn2
  L_little3/RConn2 -- cq_L_little3/LConn1
  L_little3/RConn3 -- cw_L_little3/LConn1
  ct_L_little3/RConn1 -- L_little3/LConn2
  L_middle1/RConn2 -- cq_L_middle1/LConn1
  L_middle1/RConn3 -- cw_L_middle1/LConn1
  ct_L_middle1/RConn1 -- L_middle1/LConn2
  L_middle2/RConn2 -- cq_L_middle2/LConn1
  L_middle2/RConn3 -- cw_L_middle2/LConn1
  ct_L_middle2/RConn1 -- L_middle2/LConn2
  L_middle3/RConn2 -- cq_L_middle3/LConn1
  L_middle3/RConn3 -- cw_L_middle3/LConn1
  ct_L_middle3/RConn1 -- L_middle3/LConn2
  L_ring1/RConn2 -- cq_L_ring1/LConn1
  L_ring1/RConn3 -- cw_L_ring1/LConn1
  ct_L_ring1/RConn1 -- L_ring1/LConn2
  L_ring2/RConn2 -- cq_L_ring2/LConn1
  L_ring2/RConn3 -- cw_L_ring2/LConn1
  ct_L_ring2/RConn1 -- L_ring2/LConn2
  L_ring3/RConn2 -- cq_L_ring3/LConn1
  L_ring3/RConn3 -- cw_L_ring3/LConn1
  ct_L_ring3/RConn1 -- L_ring3/LConn2
  L_scapula/RConn2 -- cq_L_scapula/LConn1
  L_scapula/RConn3 -- cw_L_scapula/LConn1
  ct_L_scapula/RConn1 -- L_scapula/LConn2
  L_shin/RConn2 -- cq_L_shin/LConn1
  L_shin/RConn3 -- cw_L_shin/LConn1
  ct_L_shin/RConn1 -- L_shin/LConn2
  L_shoulder_roll/RConn2 -- cq_L_shoulder_roll/LConn1
  L_shoulder_roll/RConn3 -- cw_L_shoulder_roll/LConn1
  ct_L_shoulder_roll/RConn1 -- L_shoulder_roll/LConn2
  L_shoulder_yaw/RConn2 -- cq_L_shoulder_yaw/LConn1
  L_shoulder_yaw/RConn3 -- cw_L_shoulder_yaw/LConn1
  ct_L_shoulder_yaw/RConn1 -- L_shoulder_yaw/LConn2
  L_thigh/RConn2 -- cq_L_thigh/LConn1
  L_thigh/RConn3 -- cw_L_thigh/LConn1
  ct_L_thigh/RConn1 -- L_thigh/LConn2
  L_thumb1/RConn2 -- cq_L_thumb1/LConn1
  L_thumb1/RConn3 -- cw_L_thumb1/LConn1
  ct_L_thumb1/RConn1 -- L_thumb1/LConn2
  L_thumb2/RConn2 -- cq_L_thumb2/LConn1
  L_thumb2/RConn3 -- cw_L_thumb2/LConn1
  ct_L_thumb2/RConn1 -- L_thumb2/LConn2
  L_thumb3/RConn2 -- cq_L_thumb3/LConn1
  L_thumb3/RConn3 -- cw_L_thumb3/LConn1
  ct_L_thumb3/RConn1 -- L_thumb3/LConn2
  L_toe/RConn2 -- cq_L_toe/LConn1
  L_toe/RConn3 -- cw_L_toe/LConn1
  ct_L_toe/RConn1 -- L_toe/LConn2
  L_upper_arm/RConn2 -- cq_L_upper_arm/LConn1
  L_upper_arm/RConn3 -- cw_L_upper_arm/LConn1
  ct_L_upper_arm/RConn1 -- L_upper_arm/LConn2
  L_wrist_roll/RConn2 -- cq_L_wrist_roll/LConn1
  L_wrist_roll/RConn3 -- cw_L_wrist_roll/LConn1
  ct_L_wrist_roll/RConn1 -- L_wrist_roll/LConn2
  L_wrist_yaw/RConn2 -- cq_L_wrist_yaw/LConn1
  L_wrist_yaw/RConn3 -- cw_L_wrist_yaw/LConn1
  ct_L_wrist_yaw/RConn1 -- L_wrist_yaw/LConn2
  R_ankle_pitch/RConn2 -- cq_R_ankle_pitch/LConn1
  R_ankle_pitch/RConn3 -- cw_R_ankle_pitch/LConn1
  ct_R_ankle_pitch/RConn1 -- R_ankle_pitch/LConn2
  R_arm_twist/RConn2 -- cq_R_arm_twist/LConn1
  R_arm_twist/RConn3 -- cw_R_arm_twist/LConn1
  ct_R_arm_twist/RConn1 -- R_arm_twist/LConn2
  R_foot/RConn2 -- cq_R_foot/LConn1
  R_foot/RConn3 -- cw_R_foot/LConn1
  ct_R_foot/RConn1 -- R_foot/LConn2
  R_forearm/RConn2 -- cq_R_forearm/LConn1
  R_forearm/RConn3 -- cw_R_forearm/LConn1
  ct_R_forearm/RConn1 -- R_forearm/LConn2
  R_forearm_twist/RConn2 -- cq_R_forearm_twist/LConn1
  R_forearm_twist/RConn3 -- cw_R_forearm_twist/LConn1
  ct_R_forearm_twist/RConn1 -- R_forearm_twist/LConn2
  R_hand/RConn2 -- cq_R_hand/LConn1
  R_hand/RConn3 -- cw_R_hand/LConn1
  ct_R_hand/RConn1 -- R_hand/LConn2
  R_hip_aux/RConn2 -- cq_R_hip_aux/LConn1
  R_hip_aux/RConn3 -- cw_R_hip_aux/LConn1
  ct_R_hip_aux/RConn1 -- R_hip_aux/LConn2
  R_hip_roll/RConn2 -- cq_R_hip_roll/LConn1
  R_hip_roll/RConn3 -- cw_R_hip_roll/LConn1
  ct_R_hip_roll/RConn1 -- R_hip_roll/LConn2
  R_hip_yaw/RConn2 -- cq_R_hip_yaw/LConn1
  R_hip_yaw/RConn3 -- cw_R_hip_yaw/LConn1
  ct_R_hip_yaw/RConn1 -- R_hip_yaw/LConn2
  R_index1/RConn2 -- cq_R_index1/LConn1
  R_index1/RConn3 -- cw_R_index1/LConn1
  ct_R_index1/RConn1 -- R_index1/LConn2
  R_index2/RConn2 -- cq_R_index2/LConn1
  R_index2/RConn3 -- cw_R_index2/LConn1
  ct_R_index2/RConn1 -- R_index2/LConn2
  R_index3/RConn2 -- cq_R_index3/LConn1
  R_index3/RConn3 -- cw_R_index3/LConn1
  ct_R_index3/RConn1 -- R_index3/LConn2
  R_little1/RConn2 -- cq_R_little1/LConn1
  R_little1/RConn3 -- cw_R_little1/LConn1
  ct_R_little1/RConn1 -- R_little1/LConn2
  R_little2/RConn2 -- cq_R_little2/LConn1
  R_little2/RConn3 -- cw_R_little2/LConn1
  ct_R_little2/RConn1 -- R_little2/LConn2
  R_little3/RConn2 -- cq_R_little3/LConn1
  R_little3/RConn3 -- cw_R_little3/LConn1
  ct_R_little3/RConn1 -- R_little3/LConn2
  R_middle1/RConn2 -- cq_R_middle1/LConn1
  R_middle1/RConn3 -- cw_R_middle1/LConn1
  ct_R_middle1/RConn1 -- R_middle1/LConn2
  R_middle2/RConn2 -- cq_R_middle2/LConn1
  R_middle2/RConn3 -- cw_R_middle2/LConn1
  ct_R_middle2/RConn1 -- R_middle2/LConn2
  R_middle3/RConn2 -- cq_R_middle3/LConn1
  R_middle3/RConn3 -- cw_R_middle3/LConn1
  ct_R_middle3/RConn1 -- R_middle3/LConn2
  R_ring1/RConn2 -- cq_R_ring1/LConn1
  R_ring1/RConn3 -- cw_R_ring1/LConn1
  ct_R_ring1/RConn1 -- R_ring1/LConn2
  R_ring2/RConn2 -- cq_R_ring2/LConn1
  R_ring2/RConn3 -- cw_R_ring2/LConn1
  ct_R_ring2/RConn1 -- R_ring2/LConn2
  R_ring3/RConn2 -- cq_R_ring3/LConn1
  R_ring3/RConn3 -- cw_R_ring3/LConn1
  ct_R_ring3/RConn1 -- R_ring3/LConn2
  R_scapula/RConn2 -- cq_R_scapula/LConn1
  R_scapula/RConn3 -- cw_R_scapula/LConn1
  ct_R_scapula/RConn1 -- R_scapula/LConn2
  R_shin/RConn2 -- cq_R_shin/LConn1
  R_shin/RConn3 -- cw_R_shin/LConn1
  ct_R_shin/RConn1 -- R_shin/LConn2
  R_shoulder_roll/RConn2 -- cq_R_shoulder_roll/LConn1
  R_shoulder_roll/RConn3 -- cw_R_shoulder_roll/LConn1
  ct_R_shoulder_roll/RConn1 -- R_shoulder_roll/LConn2
  R_shoulder_yaw/RConn2 -- cq_R_shoulder_yaw/LConn1
  R_shoulder_yaw/RConn3 -- cw_R_shoulder_yaw/LConn1
  ct_R_shoulder_yaw/RConn1 -- R_shoulder_yaw/LConn2
  R_thigh/RConn2 -- cq_R_thigh/LConn1
  R_thigh/RConn3 -- cw_R_thigh/LConn1
  ct_R_thigh/RConn1 -- R_thigh/LConn2
  R_thumb1/RConn2 -- cq_R_thumb1/LConn1
  R_thumb1/RConn3 -- cw_R_thumb1/LConn1
  ct_R_thumb1/RConn1 -- R_thumb1/LConn2
  R_thumb2/RConn2 -- cq_R_thumb2/LConn1
  R_thumb2/RConn3 -- cw_R_thumb2/LConn1
  ct_R_thumb2/RConn1 -- R_thumb2/LConn2
  R_thumb3/RConn2 -- cq_R_thumb3/LConn1
  R_thumb3/RConn3 -- cw_R_thumb3/LConn1
  ct_R_thumb3/RConn1 -- R_thumb3/LConn2
  R_toe/RConn2 -- cq_R_toe/LConn1
  R_toe/RConn3 -- cw_R_toe/LConn1
  ct_R_toe/RConn1 -- R_toe/LConn2
  R_upper_arm/RConn2 -- cq_R_upper_arm/LConn1
  R_upper_arm/RConn3 -- cw_R_upper_arm/LConn1
  ct_R_upper_arm/RConn1 -- R_upper_arm/LConn2
  R_wrist_roll/RConn2 -- cq_R_wrist_roll/LConn1
  R_wrist_roll/RConn3 -- cw_R_wrist_roll/LConn1
  ct_R_wrist_roll/RConn1 -- R_wrist_roll/LConn2
  R_wrist_yaw/RConn2 -- cq_R_wrist_yaw/LConn1
  R_wrist_yaw/RConn3 -- cw_R_wrist_yaw/LConn1
  ct_R_wrist_yaw/RConn1 -- R_wrist_yaw/LConn2
  neck_pitch/RConn2 -- cq_neck_pitch/LConn1
  neck_pitch/RConn3 -- cw_neck_pitch/LConn1
  ct_neck_pitch/RConn1 -- neck_pitch/LConn2
  neck_roll/RConn2 -- cq_neck_roll/LConn1
  neck_roll/RConn3 -- cw_neck_roll/LConn1
  ct_neck_roll/RConn1 -- neck_roll/LConn2
  neck_yaw/RConn2 -- cq_neck_yaw/LConn1
  neck_yaw/RConn3 -- cw_neck_yaw/LConn1
  ct_neck_yaw/RConn1 -- neck_yaw/LConn2
  waist_pitch/RConn2 -- cq_waist_pitch/LConn1
  waist_pitch/RConn3 -- cw_waist_pitch/LConn1
  ct_waist_pitch/RConn1 -- waist_pitch/LConn2
  waist_roll/RConn2 -- cq_waist_roll/LConn1
  waist_roll/RConn3 -- cw_waist_roll/LConn1
  ct_waist_roll/RConn1 -- waist_roll/LConn2
  waist_yaw/RConn2 -- cq_waist_yaw/LConn1
  waist_yaw/RConn3 -- cw_waist_yaw/LConn1
  ct_waist_yaw/RConn1 -- waist_yaw/LConn2
